simulink model "Lab2_Task_5_final"  (R2025a)
settings: Solver=FixedStepAuto  StartTime=0.0  StopTime=inf  RelTol=1e-3
model workspace (MAT data in the model file):
  SL_ROS_VariableLengthArrays_MaxSizes.CommonInfo.ArrayTruncateAction = 'EmitWarning'
  SL_ROS_VariableLengthArrays_MaxSizes.MsgTypeMap = containers.Map
  SL_ROS_VariableLengthArrays_MaxSizes.MsgTypeMap.serialization.keys = {'sensor_msgs/LaserScan'}
  SL_ROS_VariableLengthArrays_MaxSizes.MsgTypeMap.serialization.values{1}(1).PropertyName = 'intensities'
  SL_ROS_VariableLengthArrays_MaxSizes.MsgTypeMap.serialization.values{1}(1).DataType = 'single'
  SL_ROS_VariableLengthArrays_MaxSizes.MsgTypeMap.serialization.values{1}(1).MaxLength = 360
  SL_ROS_VariableLengthArrays_MaxSizes.MsgTypeMap.serialization.values{1}(2).PropertyName = 'ranges'
  SL_ROS_VariableLengthArrays_MaxSizes.MsgTypeMap.serialization.values{1}(2).DataType = 'single'
  SL_ROS_VariableLengthArrays_MaxSizes.MsgTypeMap.serialization.values{1}(2).MaxLength = 360
  SL_ROS_VariableLengthArrays_MaxSizes.MsgTypeMap.serialization.uniformity = 0
  SL_ROS_VariableLengthArrays_MaxSizes.MsgTypeMap.serialization.keyType = 'char'
  SL_ROS_VariableLengthArrays_MaxSizes.MsgTypeMap.serialization.valueType = 'any'
undefined symbols (not defined in the file or in its folder): angdiff, header, twist
libraries: ros2lib x4, simulink_extras x1, simulink x1
(part 1 of 2)
settings Model: Creator=scott  LastModifiedBy=abodynasser22
settings OptimizationCC: DefaultParameterBehavior=Inlined  EnhancedBackFolding=on  PassReuseOutputArgsAs=Individual arguments  ZeroExternalMemoryAtStartup=off  ZeroInternalMemoryAtStartup=off  MaxStackSize=64  OptimizeBlockOrder=speed  DifferentSizesBufferReuse=on  OptimizationCustomize=off  EfficientTunableParamExpr=on
settings DebuggingCC: ParameterTunabilityLossMsg=error
settings HardwareCC: ProdBitPerPointer=32.0  ProdBitPerSizeT=32.0  ProdBitPerPtrDiffT=32.0  ProdWordSize=32.0  ProdHWDeviceType=Intel->x86-32 (Windows32)  UseEmbeddedCoderFeatures=off
settings SFSimCC: MATLABDynamicMemAlloc=off
settings RTWCC: SystemTargetFile=ert.tlc  HardwareBoard=Robot Operating System 2 (ROS 2)  TLCOptions="-aInlineSetEventsForThisBaseRateFcn=TLC_FALSE -aSuppressMultiTaskScheduler=TLC_FALSE  -aRateBasedStepFcn=0"  TemplateMakefile=ert_default_tmf  Toolchain=Colcon Tools  TargetLang=C++  Description=Embedded Coder
settings CodeAppCC: ForceParamTrailComments=on  IgnoreCustomStorageClasses=off  OperatorAnnotations=on  SimulinkDataObjDesc=on  SFDataObjDesc=on  InsertBlockDesc=on
settings ERTTargetCC: ExtModeTransport=2.0  ExtModeAutomaticAllocSize=off  RootIOFormat=Structure reference  CodeInterfacePackaging=C++ class  SupportNonInlinedSFcns=on

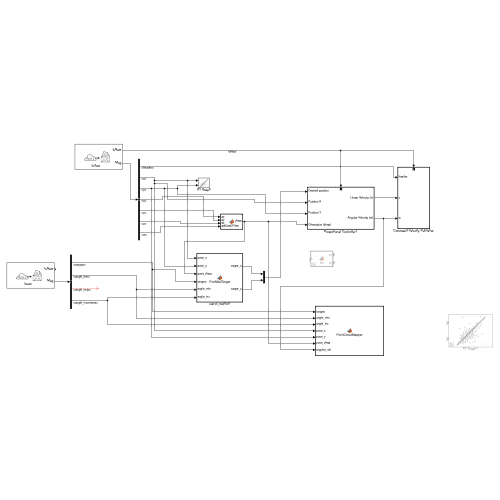
[thumbnail: Simulink's stored preview of the top-level diagram]
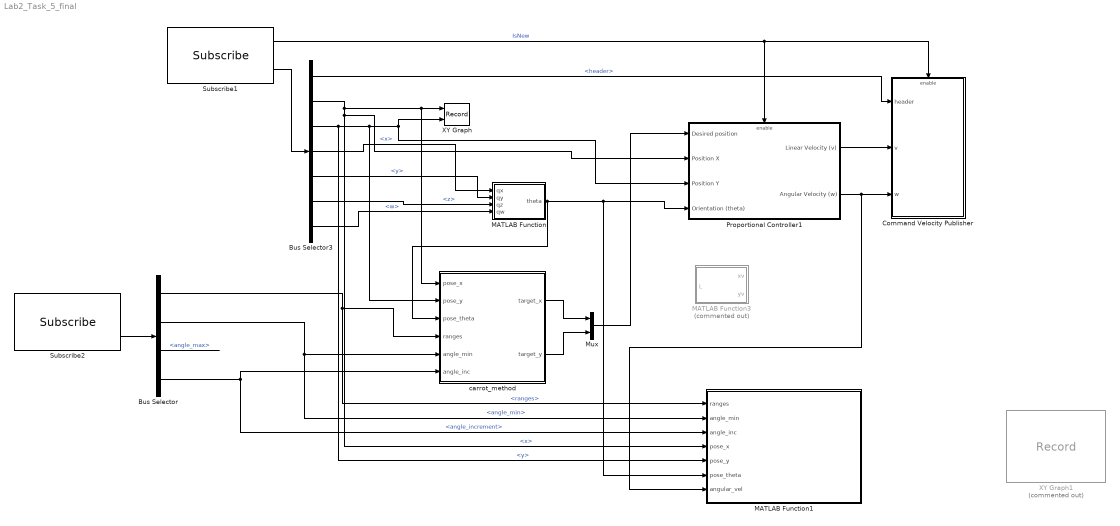
== system Lab2_Task_5_final ==
  Bus Selector : BusSelector  OutputSignals=ranges,angle_min,angle_max,angle_increment
  Bus Selector3 : BusSelector  OutputSignals=header,pose.pose.position.x,pose.pose.position.y,pose.pose.orientation.x,pose.pose.orientation.y,pose.pose.orientation.z,pose.pose.orientation.w
  Command Velocity Publisher : Subsystem
  MATLAB Function : MATLAB Function  TreatAsAtomicUnit=on
  MATLAB Function1 : MATLAB Function  TreatAsAtomicUnit=on
  MATLAB Function3 : MATLAB Function  Commented=on  TreatAsAtomicUnit=on
  Mux : Mux  Inputs=2
  Proportional Controller1 : Subsystem
  Subscribe1 : ros2lib/Subscribe  topicSource=Select from ROS network  topic=/odom  messageType=nav_msgs/Odometry  sampleTime=-1  QOSHistory=Keep last  QOSDepth=10  QOSReliability=Reliable  QOSDurability=Volatile  QOSDeadline=Inf  QOSLifespan=Inf  QOSLiveliness=Automatic  QOSLeaseDuration=Inf  QOSAvoidROSNamespaceConventions=off
  Subscribe2 : ros2lib/Subscribe  topicSource=Select from ROS network  topic=/scan  messageType=sensor_msgs/LaserScan  sampleTime=-1  QOSHistory=Keep last  QOSDepth=10  QOSReliability=Best effort  QOSDurability=Volatile  QOSDeadline=Inf  QOSLifespan=Inf  QOSLiveliness=Automatic  QOSLeaseDuration=Inf  QOSAvoidROSNamespaceConventions=off
  XY Graph : Record  NumPorts=2.0  FileSettingsInternal="{\"entries\":[{\"content\":{\"excelSettings\":{\"content\":{},\"type\":\"Streamout.ExcelSettings\"},\"parquetSettings\":{\"content\":{},\"type\":\"Streamout.ParquetSettings\"}},\"type\":\"Streamout.FileSettingStorage\",\"uuid\":\"\"}],\"packageUris\":[\"http:\\/\\/schema.mathworks.com\\/mf0\\/streamout_blocks\\/R2020a\"],\"version\":\"1.0\"}"  FrameSettings=[0, 0]  Layout=[1 1]  SignalsInternal="{\"entries\":[{\"content\":{\"signals\":[{\"content\":{\"blockPath\":[],\"dimensions\":[1],\"domain\":\"\",\"lineColor\":\"#b746ff\",\"lineWidth\":2,\"port\":1,\"signalID\":1,\"signalName\":\"<x>\"},\"type\":\"RecordBlkView.Signal\",\"uuid\":\"\"},{\"content\":{\"blockPath\":[],\"dimensions\":[1],\"domain\":\"\",\"lineColor\":\"#64d413\",\"lineWidth\":2,\"port\":2,\"signalID\":2,\"signalName\":\"<y>\"},\"type\":\"RecordBlkView.Signal\",\"uuid\":\"\"}]},\"type\":\"RecordBlkView.InputSignals\",\"uuid\":\"\"}],\"packageUris\":[\"http:\\/\\/schema.mathworks.com\\/mf0\\/streamout_blocks\\/R2020a\"],\"version\":\"1.0\"}"  VisualizationBindings="{\"xyplotplugin\":{\"info\":[{\"series\":[],\"subplotID\":1}]}}"  CompatibilityTag=XY
  XY Graph1 : Record  Commented=on  NumPorts=2.0  FileSettingsInternal="{\"entries\":[{\"content\":{\"excelSettings\":{\"content\":{},\"type\":\"Streamout.ExcelSettings\"},\"parquetSettings\":{\"content\":{},\"type\":\"Streamout.ParquetSettings\"}},\"type\":\"Streamout.FileSettingStorage\",\"uuid\":\"\"}],\"packageUris\":[\"http:\\/\\/schema.mathworks.com\\/mf0\\/streamout_blocks\\/R2020a\"],\"version\":\"1.0\"}"  FrameSettings=[0, 0]  Layout=[1 1]  SignalsInternal="{\"entries\":[{\"content\":{\"signals\":[{\"content\":{\"blockPath\":[],\"dimensions\":[360,1],\"domain\":\"\",\"hasChildren\":true,\"lineColor\":\"#d95319\",\"lineWidth\":2,\"port\":1,\"signalID\":1,\"signalName\":\"MATLAB Function1:1\"},\"type\":\"RecordBlkView.Signal\",\"uuid\":\"\"},{\"content\":{\"blockPath\":[],\"channel\":[1,1],\"dimensions\":[360,1],\"domain\":\"\",\"lineColor\":\"#edb120\",\"lineWidth\":2,\"parentID\":1,\"plots\":[ 1 ],\"port\":1,\"signalID\":2,\"signalName\":\"MATLAB Function1:1\"},\"type\":\"RecordBlkView.Signal\",\"uuid\":\"\"},{\"content\":{\"blockPath\":[],\"channel\":[2,1],\"dimensions\":[360,1],\"domain\":\"\",\"lineColor\":\"#a2142f\",\"lineWidth\":2,\"parentID\":1,\"port\":1,\"signalID\":3,\"signalName\":\"MATLAB Function1:1\"},\"type\":\"RecordBlkView.Signal\",\"uuid\":\"\"},{\"content\":{\"blockPath\":[],\"channel\":[3,1],\"dimensions\":[360,1],\"domain\":\"\",\"lineColor\":\"#139fff\",\"lineWidth\":2,\"parentID\":1,\"port\":1,\"signalID\":4,\"signalName\":\"MATLAB Function1:1\"},\"type\":\"RecordBlkView.Signal\",\"uuid\":\"\"},{\"content\":{\"blockPath\":[],\"channel\":[4,1],\"dimensions\":[360,1],\"domain\":\"\",\"lineColor\":\"#ff6929\",\"lineWidth\":2,\"parentID\":1,\"port\":1,\"signalID\":5,\"signalName\":\"MATLAB Function1:1\"},\"type\":\"RecordBlkView.Signal\",\"uuid\":\"\"},{\"content\":{\"blockPath\":[],\"channel\":[5,1],\"dimensions\":[360,1],\"domain\":\"\",\"lineColor\":\"#b746ff\",\"lineWidth\":2,\"parentID\":1,\"port\":1,\"signalID\":6,\"signalName\":\"MATLAB Function1:1\"},\"type\":\"RecordBlkView.Signal\",\"uuid\":\"\"},{\"content\":{\"blockPath\":[],\"channel\":[6,1],\"dimensions\":[360,1],\"domain\":\"\",\"lineColor\":\"#64d413\",\"lineWidth\":2,\"parentID\":1,\"port\":1,\"signalID\":7,\"signalName\":\"MATLAB Function1:1\"},\"type\":\"RecordBlkView.Signal\",\"uuid\":\"\"},{\"content\":{\"blockPath\":[],\"channel\":[7,1],\"dimensions\":[360,1],\"domain\":\"\",\"lineColor\":\"#ff13a6\",\"lineWidth\":2,\"parentID\":1,\"port\":1,\"signalID\":8,\"signalName\":\"MATLAB Function1:1\"},\"type\":\"RecordBlkView.Signal\",\"uuid\":\"\"},{\"content\":{\"blockPath\":[],\"channel\":[8,1],\"dimensions\":[360,1],\"domain\":\"\",\"lineColor\":\"#fe330a\",\"lineWidth\":2,\"parentID\":1,\"port\":1,\"signalID\":9,\"signalName\":\"MATLAB Function1:1\"},\"type\":\"RecordBlkView.Signal\",\"uuid\":\"\"},{\"content\":{\"blockPath\":[],\"channel\":[9,1],\"dimensions\":[360,1],\"domain\":\"\",\"lineColor\":\"#22b573\",\"lineWidth\":2,\"parentID\":1,\"port\":1,\"signalID\":10,\"signalName\":\"MATLAB Function1:1\"},\"type\":\"RecordBlkView.Signal\",\"uuid\":\"\"},{\"content\":{\"blockPath\":[],\"channel\":[10,1],\"dimensions\":[360,1],\"domain\":\"\",\"lineColor\":\"#0072bd\",\"lineWidth\":2,\"parentID\":1,\"port\":1,\"signalID\":11,\"signalName\":\"MATLAB Function1:1\"},\"type\":\"RecordBlkView.Signal\",\"uuid\":\"\"},{\"content\":{\"blockPath\":[],\"channel\":[11,1],\"dimensions\":[360,1],\"domain\":\"\",\"lineColor\":\"#d95319\",\"lineWidth\":2,\"parentID\":1,\"port\":1,\"signalID\":12,\"signalName\":\"MATLAB Function1:1\"},\"type\":\"RecordBlkView.Signal\",\"uuid\":\"\"},{\"content\":{\"blockPath\":[],\"channel\":[12,1],\"dimensions\":[360,1],\"domain\":\"\",\"lineColor\":\"#edb120\",\"lineWidth\":2,\"parentID\":1,\"port\":1,\"signalID\":13,\"signalName\":\"MATLAB Function1:1\"},\"type\":\"RecordBlkView.Signal\",\"uuid\":\"\"},{\"content\":{\"blockPath\":[],\"channel\":[13,1],\"dimensions\":[360,1],\"domain\":\"\",\"lineColor\":\"#7e2f8e\",\"lineWidth\":2,\"parentID\":1,\"port\":1,\"signalID\":14,\"signalName\":\"MATLAB Function1:1\"},\"type\":\"RecordBlkView.Signal\",\"uuid\":\"\"},{\"content\":{\"blockPath\":[],\"channel\":[14,1],\"dimensions\":[360,1],\"domain\":\"\",\"lineColor\":\"#77ac30\",\"lineWidth\":2,\"parentID\":1,\"port\":1,\"signalID\":15,\"signalName\":\"MATLAB Function1:1\"},\"type\":\"RecordBlkView.Signal\",\"uuid\":\"\"},{\"content\":{\"blockPath\":[],\"channel\":[15,1],\"dimensions\":[360,1],\"domain\":\"\",\"lineColor\":\"#4dbeee\",\"lineWidth\":2,\"parentID\":1,\"port\":1,\"signalID\":16,\"signalName\":\"MATLAB Function1:1\"},\"type\":\"RecordBlkView.Signal\",\"uuid\":\"\"},{\"content\":{\"blockPath\":[],\"channel\":[16,1],\"dimensions\":[360,1],\"domain\":\"\",\"lineColor\":\"#a2142f\",\"lineWidth\":2,\"parentID\":1,\"port\":1,\"signalID\":17,\"signalName\":\"MATLAB Function1:1\"},\"type\":\"RecordBlkView.Signal\",\"uuid\":\"\"},{\"content\":{\"blockPath\":[],\"channel\":[17,1],\"dimensions\":[360,1],\"domain\":\"\",\"lineColor\":\"#139fff\",\"lineWidth\":2,\"parentID\":1,\"port\":1,\"signalID\":18,\"signalName\":\"MATLAB Function1:1\"},\"type\":\"RecordBlkView.Signal\",\"uuid\":\"\"},{\"content\":{\"blockPath\":[],\"channel\":[18,1],\"dimensions\":[360,1],\"domain\":\"\",\"lineColor\":\"#ff6929\",\"lineWidth\":2,\"parentID\":1,\"port\":1,\"signalID\":19,\"signalName\":\"MATLAB Function1:1\"},\"type\":\"RecordBlkView.Signal\",\"uuid\":\"\"},{\"content\":{\"blockPath\":[],\"channel\":[19,1],\"dimensions\":[360,1],\"domain\":\"\",\"lineColor\":\"#b746ff\",\"lineWidth\":2,\"parentID\":1,\"port\":1,\"signalID\":20,\"signalName\":\"MATLAB Function1:1\"},\"type\":\"RecordBlkView.Signal\",\"uuid\":\"\"},{\"content\":{\"blockPath\":[],\"channel\":[20,1],\"dimensions\":[360,1],\"domain\":\"\",\"lineColor\":\"#64d413\",\"lineWidth\":2,\"parentID\":1,\"port\":1,\"signalID\":21,\"signalName\":\"MATLAB Function1:1\"},\"type\":\"RecordBlkView.Signal\",\"uuid\":\"\"},{\"content\":{\"blockPath\":[],\"channel\":[21,1],\"dimensions\":[360,1],\"domain\":\"\",\"lineColor\":\"#ff13a6\",\"lineWidth\":2,\"parentID\":1,\"port\":1,\"signalID\":22,\"signalName\":\"MATLAB Function1:1\"},\"type\":\"RecordBlkView.Signal\",\"uuid\":\"\"},{\"content\":{\"blockPath\":[],\"channel\":[22,1],\"dimensions\":[360,1],\"domain\":\"\",\"lineColor\":\"#fe330a\",\"lineWidth\":2,\"parentID\":1,\"port\":1,\"signalID\":23,\"signalName\":\"MATLAB Function1:1\"},\"type\":\"RecordBlkView.Signal\",\"uuid\":\"\"},{\"content\":{\"blockPath\":[],\"channel\":[23,1],\"dimensions\":[360,1],\"domain\":\"\",\"lineColor\":\"#22b573\",\"lineWidth\":2,\"parentID\":1,\"port\":1,\"signalID\":24,\"signalName\":\"MATLAB Function1:1\"},\"type\":\"RecordBlkView.Signal\",\"uuid\":\"\"},{\"content\":{\"blockPath\":[],\"channel\":[24,1],\"dimensions\":[360,1],\"domain\":\"\",\"lineColor\":\"#0072bd\",\"lineWidth\":2,\"parentID\":1,\"port\":1,\"signalID\":25,\"signalName\":\"MATLAB Function1:1\"},\"type\":\"RecordBlkView.Signal\",\"uuid\":\"\"},{\"content\":{\"blockPath\":[],\"channel\":[25,1],\"dimensions\":[360,1],\"domain\":\"\",\"lineColor\":\"#d95319\",\"lineWidth\":2,\"parentID\":1,\"port\":1,\"signalID\":26,\"signalName\":\"MATLAB Function1:1\"},\"type\":\"RecordBlkView.Signal\",\"uuid\":\"\"},{\"content\":{\"blockPath\":[],\"channel\":[26,1],\"dimensions\":[360,1],\"domain\":\"\",\"lineColor\":\"#edb120\",\"lineWidth\":2,\"parentID\":1,\"port\":1,\"signalID\":27,\"signalName\":\"MATLAB Function1:1\"},\"type\":\"RecordBlkView.Signal\",\"uuid\":\"\"},{\"content\":{\"blockPath\":[],\"channel\":[27,1],\"dimensions\":[360,1],\"domain\":\"\",\"lineColor\":\"#7e2f8e\",\"lineWidth\":2,\"parentID\":1,\"port\":1,\"signalID\":28,\"signalName\":\"MATLAB Function1:1\"},\"type\":\"RecordBlkView.Signal\",\"uuid\":\"\"},{\"content\":{\"blockPath\":[],\"channel\":[28,1],\"dimensions\":[360,1],\"domain\":\"\",\"lineColor\":\"#77ac30\",\"lineWidth\":2,\"parentID\":1,\"port\":1,\"signalID\":29,\"signalName\":\"MATLAB Function1:1\"},\"type\":\"RecordBlkView.Signal\",\"uuid\":\"\"},{\"content\":{\"blockPath\":[],\"channel\":[29,1],\"dimensions\":[360,1],\"domain\":\"\",\"lineColor\":\"#4dbeee\",\"lineWidth\":2,\"parentID\":1,\"port\":1,\"signalID\":30,\"signalName\":\"MATLAB Function1:1\"},\"type\":\"RecordBlkView.Signal\",\"uuid\":\"\"},{\"content\":{\"blockPath\":[],\"channel\":[30,1],\"dimensions\":[360,1],\"domain\":\"\",\"lineColor\":\"#a2142f\",\"lineWidth\":2,\"parentID\":1,\"port\":1,\"signalID\":31,\"signalName\":\"MATLAB Function1:1\"},\"type\":\"RecordBlkView.Signal\",\"uuid\":\"\"},{\"content\":{\"blockPath\":[],\"channel\":[31,1],\"dimensions\":[360,1],\"domain\":\"\",\"lineColor\":\"#139fff\",\"lineWidth\":2,\"parentID\":1,\"port\":1,\"signalID\":32,\"signalName\":\"MATLAB Function1:1\"},\"type\":\"RecordBlkView.Signal\",\"uuid\":\"\"},{\"content\":{\"blockPath\":[],\"channel\":[32,1],\"dimensions\":[360,1],\"domain\":\"\",\"lineColor\":\"#ff6929\",\"lineWidth\":2,\"parentID\":1,\"port\":1,\"signalID\":33,\"signalName\":\"MATLAB Function1:1\"},\"type\":\"RecordBlkView.Signal\",\"uuid\":\"\"},{\"content\":{\"blockPath\":[],\"channel\":[33,1],\"dimensions\":[360,1],\"domain\":\"\",\"lineColor\":\"#b746ff\",\"lineWidth\":2,\"parentID\":1,\"port\":1,\"signalID\":34,\"signalName\":\"MATLAB Function1:1\"},\"type\":\"RecordBlkView.Signal\",\"uuid\":\"\"},{\"content\":{\"blockPath\":[],\"channel\":[34,1],\"dimensions\":[360,1],\"domain\":\"\",\"lineColor\":\"#64d413\",\"lineWidth\":2,\"parentID\":1,\"port\":1,\"signalID\":35,\"signalName\":\"MATLAB Function1:1\"},\"type\":\"RecordBlkView.Signal\",\"uuid\":\"\"},{\"content\":{\"blockPath\":[],\"channel\":[35,1],\"dimensions\":[360,1],\"domain\":\"\",\"lineColor\":\"#ff13a6\",\"lineWidth\":2,\"parentID\":1,\"port\":1,\"signalID\":36,\"signalName\":\"MATLAB Function1:1\"},\"type\":\"RecordBlkView.Signal\",\"uuid\":\"\"},{\"content\":{\"blockPath\":[],\"channel\":[36,1],\"dimensions\":[360,1],\"domain\":\"\",\"lineColor\":\"#fe330a\",\"lineWidth\":2,\"parentID\":1,\"port\":1,\"signalID\":37,\"signalName\":\"MATLAB Function1:1\"},\"type\":\"RecordBlkView.Signal\",\"uuid\":\"\"},{\"content\":{\"blockPath\":[],\"channel\":[37,1],\"dimensions\":[360,1],\"domain\":\"\",\"lineColor\":\"#22b573\",\"lineWidth\":2,\"parentID\":1,\"port\":1,\"signalID\":38,\"signalName\":\"MATLAB Function1:1\"},\"type\":\"RecordBlkView.Signal\",\"uuid\":\"\"},{\"content\":{\"blockPath\":[],\"channel\":[38,1],\"dimensions\":[360,1],\"domain\":\"\",\"lineColor\":\"#0072bd\",\"lineWidth\":2,\"parentID\":1,\"port\":1,\"signalID\":39,\"signalName\":\"MATLAB Function1:1\"},\"type\":\"RecordBlkView.Signal\",\"uuid\":\"\"},{\"content\":{\"blockPath\":[],\"channel\":[39,1],\"dimensions\":[360,1],\"domain\":\"\",\"lineColor\":\"#d95319\",\"lineWidth\":2,\"parentID\":1,\"port\":1,\"signalID\":40,\"signalName\":\"MATLAB Function1:1\"},\"type\":\"RecordBlkView.Signal\",\"uuid\":\"\"},{\"content\":{\"blockPath\":[],\"channel\":[40,1],\"dimensions\":[360,1],\"domain\":\"\",\"lineColor\":\"#edb120\",\"lineWidth\":2,\"parentID\":1,\"port\":1,\"signalID\":41,\"signalName\":\"MATLAB Function1:1\"},\"type\":\"RecordBlkView.Signal\",\"uuid\":\"\"},{\"content\":{\"blockPath\":[],\"channel\":[41,1],\"dimensions\":[360,1],\"domain\":\"\",\"lineColor\":\"#7e2f8e\",\"lineWidth\":2,\"parentID\":1,\"port\":1,\"signalID\":42,\"signalName\":\"MATLAB Function1:1\"},\"type\":\"RecordBlkView.Signal\",\"uuid\":\"\"},{\"content\":{\"blockPath\":[],\"channel\":[42,1],\"dimensions\":[360,1],\"domain\":\"\",\"lineColor\":\"#77ac30\",\"lineWidth\":2,\"parentID\":1,\"port\":1,\"signalID\":43,\"signalName\":\"MATLAB Function1:1\"},\"type\":\"RecordBlkView.Signal\",\"uuid\":\"\"},{\"content\":{\"blockPath\":[],\"channel\":[43,1],\"dimensions\":[360,1],\"domain\":\"\",\"lineColor\":\"#4dbeee\",\"lineWidth\":2,\"parentID\":1,\"port\":1,\"signalID\":44,\"signalName\":\"MATLAB Function1:1\"},\"type\":\"RecordBlkView.Signal\",\"uuid\":\"\"},{\"content\":{\"blockPath\":[],\"channel\":[44,1],\"dimensions\":[360,1],\"domain\":\"\",\"lineColor\":\"#a2142f\",\"lineWidth\":2,\"parentID\":1,\"port\":1,\"signalID\":45,\"signalName\":\"MATLAB Function1:1\"},\"type\":\"RecordBlkView.Signal\",\"uuid\":\"\"},{\"content\":{\"blockPath\":[],\"channel\":[45,1],\"dimensions\":[360,1],\"domain\":\"\",\"lineColor\":\"#139fff\",\"lineWidth\":2,\"parentID\":1,\"port\":1,\"signalID\":46,\"signalName\":\"MATLAB Function1:1\"},\"type\":\"RecordBlkView.Signal\",\"uuid\":\"\"},{\"content\":{\"blockPath\":[],\"channel\":[46,1],\"dimensions\":[360,1],\"domain\":\"\",\"lineColor\":\"#ff6929\",\"lineWidth\":2,\"parentID\":1,\"port\":1,\"signalID\":47,\"signalName\":\"MATLAB Function1:1\"},\"type\":\"RecordBlkView.Signal\",\"uuid\":\"\"},{\"content\":{\"blockPath\":[],\"channel\":[47,1],\"dimensions\":[360,1],\"domain\":\"\",\"lineColor\":\"#b746ff\",\"lineWidth\":2,\"parentID\":1,\"port\":1,\"signalID\":48,\"signalName\":\"MATLAB Function1:1\"},\"type\":\"RecordBlkView.Signal\",\"uuid\":\"\"},{\"content\":{\"blockPath\":[],\"channel\":[48,1],\"dimensions\":[360,1],\"domain\":\"\",\"lineColor\":\"#64d413\",\"lineWidth\":2,\"parentID\":1,\"port\":1,\"signalID\":49,\"signalName\":\"MATLAB Function1:1\"},\"type\":\"RecordBlkView.Signal\",\"uuid\":\"\"},{\"content\":{\"blockPath\":[],\"channel\":[49,1],\"dimensions\":[360,1],\"domain\":\"\",\"lineColor\":\"#ff13a6\",\"lineWidth\":2,\"parentID\":1,\"port\":1,\"signalID\":50,\"signalName\":\"MATLAB Function1:1\"},\"type\":\"RecordBlkView.Signal\",\"uuid\":\"\"},{\"content\":{\"blockPath\":[],\"channel\":[50,1],\"dimensions\":[360,1],\"domain\":\"\",\"lineColor\":\"#fe330a\",\"lineWidth\":2,\"parentID\":1,\"port\":1,\"signalID\":51,\"signalName\":\"MATLAB Function1:1\"},\"type\":\"RecordBlkView.Signal\",\"uuid\":\"\"},{\"content\":{\"blockPath\":[],\"channel\":[51,1],\"dimensions\":[360,1],\"domain\":\"\",\"lineColor\":\"#22b573\",\"lineWidth\":2,\"parentID\":1,\"port\":1,\"signalID\":52,\"signalName\":\"MATLAB Function1:1\"},\"type\":\"RecordBlkView.Signal\",\"uuid\":\"\"},{\"content\":{\"blockPath\":[],\"channel\":[52,1],\"dimensions\":[360,1],\"domain\":\"\",\"lineColor\":\"#0072bd\",\"lineWidth\":2,\"parentID\":1,\"port\":1,\"signalID\":53,\"signalName\":\"MATLAB Function1:1\"},\"type\":\"RecordBlkView.Signal\",\"uuid\":\"\"},{\"content\":{\"blockPath\":[],\"channel\":[53,1],\"dimensions\":[360,1],\"domain\":\"\",\"lineColor\":\"#d95319\",\"lineWidth\":2,\"parentID\":1,\"port\":1,\"signalID\":54,\"signalName\":\"MATLAB Function1:1\"},\"type\":\"RecordBlkView.Signal\",\"uuid\":\"\"},{\"content\":{\"blockPath\":[],\"channel\":[54,1],\"dimensions\":[360,1],\"domain\":\"\",\"lineColor\":\"#edb120\",\"lineWidth\":2,\"parentID\":1,\"port\":1,\"signalID\":55,\"signalName\":\"MATLAB Function1:1\"},\"type\":\"RecordBlkView.Signal\",\"uuid\":\"\"},{\"content\":{\"blockPath\":[],\"channel\":[55,1],\"dimensions\":[360,1],\"domain\":\"\",\"lineColor\":\"#7e2f8e\",\"lineWidth\":2,\"parentID\":1,\"port\":1,\"signalID\":56,\"signalName\":\"MATLAB Function1:1\"},\"type\":\"RecordBlkView.Signal\",\"uuid\":\"\"},{\"content\":{\"blockPath\":[],\"channel\":[56,1],\"dimensions\":[360,1],\"domain\":\"\",\"lineColor\":\"#77ac30\",\"lineWidth\":2,\"parentID\":1,\"port\":1,\"signalID\":57,\"signalName\":\"MATLAB Function1:1\"},\"type\":\"RecordBlkView.Signal\",\"uuid\":\"\"},{\"content\":{\"blockPath\":[],\"channel\":[57,1],\"dimensions\":[360,1],\"domain\":\"\",\"lineColor\":\"#4dbeee\",\"lineWidth\":2,\"parentID\":1,\"port\":1,\"signalID\":58,\"signalName\":\"MATLAB Function1:1\"},\"type\":\"RecordBlkView.Signal\",\"uuid\":\"\"},{\"content\":{\"blockPath\":[],\"channel\":[58,1],\"dimensions\":[360,1],\"domain\":\"\",\"lineColor\":\"#a2142f\",\"lineWidth\":2,\"parentID\":1,\"port\":1,\"signalID\":59,\"signalName\":\"MATLAB Function1:1\"},\"type\":\"RecordBlkView.Signal\",\"uuid\":\"\"},{\"content\":{\"blockPath\":[],\"channel\":[59,1],\"dimensions\":[360,1],\"domain\":\"\",\"lineColor\":\"#139fff\",\"lineWidth\":2,\"parentID\":1,\"port\":1,\"signalID\":60,\"signalName\":\"MATLAB Function1:1\"},\"type\":\"RecordBlkView.Signal\",\"uuid\":\"\"},{\"content\":{\"blockPath\":[],\"channel\":[60,1],\"dimensions\":[360,1],\"domain\":\"\",\"lineColor\":\"#ff6929\",\"lineWidth\":2,\"parentID\":1,\"port\":1,\"signalID\":61,\"signalName\":\"MATLAB Function1:1\"},\"type\":\"RecordBlkView.Signal\",\"uuid\":\"\"},{\"content\":{\"blockPath\":[],\"channel\":[61,1],\"dimensions\":[360,1],\"domain\":\"\",\"lineColor\":\"#b746ff\",\"lineWidth\":2,\"parentID\":1,\"port\":1,\"signalID\":62,\"signalName\":\"MATLAB Function1:1\"},\"type\":\"RecordBlkView.Signal\",\"uuid\":\"\"},{\"content\":{\"blockPath\":[],\"channel\":[62,1],\"dimensions\":[360,1],\"domain\":\"\",\"lineColor\":\"#64d413\",\"lineWidth\":2,\"parentID\":1,\"port\":1,\"signalID\":63,\"signalName\":\"MATLAB Function1:1\"},\"type\":\"RecordBlkView.Signal\",\"uuid\":\"\"},{\"content\":{\"blockPath\":[],\"channel\":[63,1],\"dimensions\":[360,1],\"domain\":\"\",\"lineColor\":\"#ff13a6\",\"lineWidth\":2,\"parentID\":1,\"port\":1,\"signalID\":64,\"signalName\":\"MATLAB Function1:1\"},\"type\":\"RecordBlkView.Signal\",\"uuid\":\"\"},{\"content\":{\"blockPath\":[],\"channel\":[64,1],\"dimensions\":[360,1],\"domain\":\"\",\"lineColor\":\"#fe330a\",\"lineWidth\":2,\"parentID\":1,\"port\":1,\"signalID\":65,\"signalName\":\"MATLAB Function1:1\"},\"type\":\"RecordBlkView.Signal\",\"uuid\":\"\"},{\"content\":{\"blockPath\":[],\"channel\":[65,1],\"dimensions\":[360,1],\"domain\":\"\",\"lineColor\":\"#22b573\",\"lineWidth\":2,\"parentID\":1,\"port\":1,\"signalID\":66,\"signalName\":\"MATLAB Function1:1\"},\"type\":\"RecordBlkView.Signal\",\"uuid\":\"\"},{\"content\":{\"blockPath\":[],\"channel\":[66,1],\"dimensions\":[360,1],\"domain\":\"\",\"lineColor\":\"#0072bd\",\"lineWidth\":2,\"parentID\":1,\"port\":1,\"signalID\":67,\"signalName\":\"MATLAB Function1:1\"},\"type\":\"RecordBlkView.Signal\",\"uuid\":\"\"},{\"content\":{\"blockPath\":[],\"channel\":[67,1],\"dimensions\":[360,1],\"domain\":\"\",\"lineColor\":\"#d95319\",\"lineWidth\":2,\"parentID\":1,\"port\":1,\"signalID\":68,\"signalName\":\"MATLAB Function1:1\"},\"type\":\"RecordBlkView.Signal\",\"uuid\":\"\"},{\"content\":{\"blockPath\":[],\"channel\":[68,1],\"dimensions\":[360,1],\"domain\":\"\",\"lineColor\":\"#edb120\",\"lineWidth\":2,\"parentID\":1,\"port\":1,\"signalID\":69,\"signalName\":\"MATLAB Function1:1\"},\"type\":\"RecordBlkView.Signal\",\"uuid\":\"\"},{\"content\":{\"blockPath\":[],\"channel\":[69,1],\"dimensions\":[360,1],\"domain\":\"\",\"lineColor\":\"#7e2f8e\",\"lineWidth\":2,\"parentID\":1,\"port\":1,\"signalID\":70,\"signalName\":\"MATLAB Function1:1\"},\"type\":\"RecordBlkView.Signal\",\"uuid\":\"\"},{\"content\":{\"blockPath\":[],\"channel\":[70,1],\"dimensions\":[360,1],\"domain\":\"\",\"lineColor\":\"#77ac30\",\"lineWidth\":2,\"parentID\":1,\"port\":1,\"signalID\":71,\"signalName\":\"MATLAB Function1:1\"},\"type\":\"RecordBlkView.Signal\",\"uuid\":\"\"},{\"content\":{\"blockPath\":[],\"channel\":[71,1],\"dimensions\":[360,1],\"domain\":\"\",\"lineColor\":\"#4dbeee\",\"lineWidth\":2,\"parentID\":1,\"port\":1,\"signalID\":72,\"signalName\":\"MATLAB Function1:1\"},\"type\":\"RecordBlkView.Signal\",\"uuid\":\"\"},{\"content\":{\"blockPath\":[],\"channel\":[72,1],\"dimensions\":[360,1],\"domain\":\"\",\"lineColor\":\"#a2142f\",\"lineWidth\":2,\"parentID\":1,\"port\":1,\"signalID\":73,\"signalName\":\"MATLAB Function1:1\"},\"type\":\"RecordBlkView.Signal\",\"uuid\":\"\"},{\"content\":{\"blockPath\":[],\"channel\":[73,1],\"dimensions\":[360,1],\"domain\":\"\",\"lineColor\":\"#139fff\",\"lineWidth\":2,\"parentID\":1,\"port\":1,\"signalID\":74,\"signalName\":\"MATLAB Function1:1\"},\"type\":\"RecordBlkView.Signal\",\"uuid\":\"\"},{\"content\":{\"blockPath\":[],\"channel\":[74,1],\"dimensions\":[360,1],\"domain\":\"\",\"lineColor\":\"#ff6929\",\"lineWidth\":2,\"parentID\":1,\"port\":1,\"signalID\":75,\"signalName\":\"MATLAB Function1:1\"},\"type\":\"RecordBlkView.Signal\",\"uuid\":\"\"},{\"content\":{\"blockPath\":[],\"channel\":[75,1],\"dimensions\":[360,1],\"domain\":\"\",\"lineColor\":\"#b746ff\",\"lineWidth\":2,\"parentID\":1,\"port\":1,\"signalID\":76,\"signalName\":\"MATLAB Function1:1\"},\"type\":\"RecordBlkView.Signal\",\"uuid\":\"\"},{\"content\":{\"blockPath\":[],\"channel\":[76,1],\"dimensions\":[360,1],\"domain\":\"\",\"lineColor\":\"#64d413\",\"lineWidth\":2,\"parentID\":1,\"port\":1,\"signalID\":77,\"signalName\":\"MATLAB Function1:1\"},\"type\":\"RecordBlkView.Signal\",\"uuid\":\"\"},{\"content\":{\"blockPath\":[],\"channel\":[77,1],\"dimensions\":[360,1],\"domain\":\"\",\"lineColor\":\"#ff13a6\",\"lineWidth\":2,\"parentID\":1,\"port\":1,\"signalID\":78,\"signalName\":\"MATLAB Function1:1\"},\"type\":\"RecordBlkView.Signal\",\"uuid\":\"\"},{\"content\":{\"blockPath\":[],\"channel\":[78,1],\"dimensions\":[360,1],\"domain\":\"\",\"lineColor\":\"#fe330a\",\"lineWidth\":2,\"parentID\":1,\"port\":1,\"signalID\":79,\"signalName\":\"MATLAB Function1:1\"},\"type\":\"RecordBlkView.Signal\",\"uuid\":\"\"},{\"content\":{\"blockPath\":[],\"channel\":[79,1],\"dimensions\":[360,1],\"domain\":\"\",\"lineColor\":\"#22b573\",\"lineWidth\":2,\"parentID\":1,\"port\":1,\"signalID\":80,\"signalName\":\"MATLAB Function1:1\"},\"type\":\"RecordBlkView.Signal\",\"uuid\":\"\"},{\"content\":{\"blockPath\":[],\"channel\":[80,1],\"dimensions\":[360,1],\"domain\":\"\",\"lineColor\":\"#0072bd\",\"lineWidth\":2,\"parentID\":1,\"port\":1,\"signalID\":81,\"signalName\":\"MATLAB Function1:1\"},\"type\":\"RecordBlkView.Signal\",\"uuid\":\"\"},{\"content\":{\"blockPath\":[],\"channel\":[81,1],\"dimensions\":[360,1],\"domain\":\"\",\"lineColor\":\"#d95319\",\"lineWidth\":2,\"parentID\":1,\"port\":1,\"signalID\":82,\"signalName\":\"MATLAB Function1:1\"},\"type\":\"RecordBlkView.Signal\",\"uuid\":\"\"},{\"content\":{\"blockPath\":[],\"channel\":[82,1],\"dimensions\":[360,1],\"domain\":\"\",\"lineColor\":\"#edb120\",\"lineWidth\":2,\"parentID\":1,\"port\":1,\"signalID\":83,\"signalName\":\"MATLAB Function1:1\"},\"type\":\"RecordBlkView.Signal\",\"uuid\":\"\"},{\"content\":{\"blockPath\":[],\"channel\":[83,1],\"dimensions\":[360,1],\"domain\":\"\",\"lineColor\":\"#7e2f8e\",\"lineWidth\":2,\"parentID\":1,\"port\":1,\"signalID\":84,\"signalName\":\"MATLAB Function1:1\"},\"type\":\"RecordBlkView.Signal\",\"uuid\":\"\"},{\"content\":{\"blockPath\":[],\"channel\":[84,1],\"dimensions\":[360,1],\"domain\":\"\",\"lineColor\":\"#77ac30\",\"lineWidth\":2,\"parentID\":1,\"port\":1,\"signalID\":85,\"signalName\":\"MATLAB Function1:1\"},\"type\":\"RecordBlkView.Signal\",\"uuid\":\"\"},{\"content\":{\"blockPath\":[],\"channel\":[85,1],\"dimensions\":[360,1],\"domain\":\"\",\"lineColor\":\"#4dbeee\",\"lineWidth\":2,\"parentID\":1,\"port\":1,\"signalID\":86,\"signalName\":\"MATLAB Function1:1\"},\"type\":\"RecordBlkView.Signal\",\"uuid\":\"\"},{\"content\":{\"blockPath\":[],\"channel\":[86,1],\"dimensions\":[360,1],\"domain\":\"\",\"lineColor\":\"#a2142f\",\"lineWidth\":2,\"parentID\":1,\"port\":1,\"signalID\":87,\"signalName\":\"MATLAB Function1:1\"},\"type\":\"RecordBlkView.Signal\",\"uuid\":\"\"},{\"content\":{\"blockPath\":[],\"channel\":[87,1],\"dimensions\":[360,1],\"domain\":\"\",\"lineColor\":\"#139fff\",\"lineWidth\":2,\"parentID\":1,\"port\":1,\"signalID\":88,\"signalName\":\"MATLAB Function1:1\"},\"type\":\"RecordBlkView.Signal\",\"uuid\":\"\"},{\"content\":{\"blockPath\":[],\"channel\":[88,1],\"dimensions\":[360,1],\"domain\":\"\",\"lineColor\":\"#ff6929\",\"lineWidth\":2,\"parentID\":1,\"port\":1,\"signalID\":89,\"signalName\":\"MATLAB Function1:1\"},\"type\":\"RecordBlkView.Signal\",\"uuid\":\"\"},{\"content\":{\"blockPath\":[],\"channel\":[89,1],\"dimensions\":[360,1],\"domain\":\"\",\"lineColor\":\"#b746ff\",\"lineWidth\":2,\"parentID\":1,\"port\":1,\"signalID\":90,\"signalName\":\"MATLAB Function1:1\"},\"type\":\"RecordBlkView.Signal\",\"uuid\":\"\"},{\"content\":{\"blockPath\":[],\"channel\":[90,1],\"dimensions\":[360,1],\"domain\":\"\",\"lineColor\":\"#64d413\",\"lineWidth\":2,\"parentID\":1,\"port\":1,\"signalID\":91,\"signalName\":\"MATLAB Function1:1\"},\"type\":\"RecordBlkView.Signal\",\"uuid\":\"\"},{\"content\":{\"blockPath\":[],\"channel\":[91,1],\"dimensions\":[360,1],\"domain\":\"\",\"lineColor\":\"#ff13a6\",\"lineWidth\":2,\"parentID\":1,\"port\":1,\"signalID\":92,\"signalName\":\"MATLAB Function1:1\"},\"type\":\"RecordBlkView.Signal\",\"uuid\":\"\"},{\"content\":{\"blockPath\":[],\"channel\":[92,1],\"dimensions\":[360,1],\"domain\":\"\",\"lineColor\":\"#fe330a\",\"lineWidth\":2,\"parentID\":1,\"port\":1,\"signalID\":93,\"signalName\":\"MATLAB Function1:1\"},\"type\":\"RecordBlkView.Signal\",\"uuid\":\"\"},{\"content\":{\"blockPath\":[],\"channel\":[93,1],\"dimensions\":[360,1],\"domain\":\"\",\"lineColor\":\"#22b573\",\"lineWidth\":2,\"parentID\":1,\"port\":1,\"signalID\":94,\"signalName\":\"MATLAB Function1:1\"},\"type\":\"RecordBlkView.Signal\",\"uuid\":\"\"},{\"content\":{\"blockPath\":[],\"channel\":[94,1],\"dimensions\":[360,1],\"domain\":\"\",\"lineColor\":\"#0072bd\",\"lineWidth\":2,\"parentID\":1,\"port\":1,\"signalID\":95,\"signalName\":\"MATLAB Function1:1\"},\"type\":\"RecordBlkView.Signal\",\"uuid\":\"\"},{\"content\":{\"blockPath\":[],\"channel\":[95,1],\"dimensions\":[360,1],\"domain\":\"\",\"lineColor\":\"#d95319\",\"lineWidth\":2,\"parentID\":1,\"port\":1,\"signalID\":96,\"signalName\":\"MATLAB Function1:1\"},\"type\":\"RecordBlkView.Signal\",\"uuid\":\"\"},{\"content\":{\"blockPath\":[],\"channel\":[96,1],\"dimensions\":[360,1],\"domain\":\"\",\"lineColor\":\"#edb120\",\"lineWidth\":2,\"parentID\":1,\"port\":1,\"signalID\":97,\"signalName\":\"MATLAB Function1:1\"},\"type\":\"RecordBlkView.Signal\",\"uuid\":\"\"},{\"content\":{\"blockPath\":[],\"channel\":[97,1],\"dimensions\":[360,1],\"domain\":\"\",\"lineColor\":\"#7e2f8e\",\"lineWidth\":2,\"parentID\":1,\"port\":1,\"signalID\":98,\"signalName\":\"MATLAB Function1:1\"},\"type\":\"RecordBlkView.Signal\",\"uuid\":\"\"},{\"content\":{\"blockPath\":[],\"channel\":[98,1],\"dimensions\":[360,1],\"domain\":\"\",\"lineColor\":\"#77ac30\",\"lineWidth\":2,\"parentID\":1,\"port\":1,\"signalID\":99,\"signalName\":\"MATLAB Function1:1\"},\"type\":\"RecordBlkView.Signal\",\"uuid\":\"\"},{\"content\":{\"blockPath\":[],\"channel\":[99,1],\"dimensions\":[360,1],\"domain\":\"\",\"lineColor\":\"#4dbeee\",\"lineWidth\":2,\"parentID\":1,\"port\":1,\"signalID\":100,\"signalName\":\"MATLAB Function1:1\"},\"type\":\"RecordBlkView.Signal\",\"uuid\":\"\"},{\"content\":{\"blockPath\":[],\"channel\":[100,1],\"dimensions\":[360,1],\"domain\":\"\",\"lineColor\":\"#a2142f\",\"lineWidth\":2,\"parentID\":1,\"port\":1,\"signalID\":101,\"signalName\":\"MATLAB Function1:1\"},\"type\":\"RecordBlkView.Signal\",\"uuid\":\"\"},{\"content\":{\"blockPath\":[],\"channel\":[101,1],\"dimensions\":[360,1],\"domain\":\"\",\"lineColor\":\"#139fff\",\"lineWidth\":2,\"parentID\":1,\"port\":1,\"signalID\":102,\"signalName\":\"MATLAB Function1:1\"},\"type\":\"RecordBlkView.Signal\",\"uuid\":\"\"},{\"content\":{\"blockPath\":[],\"channel\":[102,1],\"dimensions\":[360,1],\"domain\":\"\",\"lineColor\":\"#ff6929\",\"lineWidth\":2,\"parentID\":1,\"port\":1,\"signalID\":103,\"signalName\":\"MATLAB Function1:1\"},\"type\":\"RecordBlkView.Signal\",\"uuid\":\"\"},{\"content\":{\"blockPath\":[],\"channel\":[103,1],\"dimensions\":[360,1],\"domain\":\"\",\"lineColor\":\"#b746ff\",\"lineWidth\":2,\"parentID\":1,\"port\":1,\"signalID\":104,\"signalName\":\"MATLAB Function1:1\"},\"type\":\"RecordBlkView.Signal\",\"uuid\":\"\"},{\"content\":{\"blockPath\":[],\"channel\":[104,1],\"dimensions\":[360,1],\"domain\":\"\",\"lineColor\":\"#64d413\",\"lineWidth\":2,\"parentID\":1,\"port\":1,\"signalID\":105,\"signalName\":\"MATLAB Function1:1\"},\"type\":\"RecordBlkView.Signal\",\"uuid\":\"\"},{\"content\":{\"blockPath\":[],\"channel\":[105,1],\"dimensions\":[360,1],\"domain\":\"\",\"lineColor\":\"#ff13a6\",\"lineWidth\":2,\"parentID\":1,\"port\":1,\"signalID\":106,\"signalName\":\"MATLAB Function1:1\"},\"type\":\"RecordBlkView.Signal\",\"uuid\":\"\"},{\"content\":{\"blockPath\":[],\"channel\":[106,1],\"dimensions\":[360,1],\"domain\":\"\",\"lineColor\":\"#fe330a\",\"lineWidth\":2,\"parentID\":1,\"port\":1,\"signalID\":107,\"signalName\":\"MATLAB Function1:1\"},\"type\":\"RecordBlkView.Signal\",\"uuid\":\"\"},{\"content\":{\"blockPath\":[],\"channel\":[107,1],\"dimensions\":[360,1],\"domain\":\"\",\"lineColor\":\"#22b573\",\"lineWidth\":2,\"parentID\":1,\"port\":1,\"signalID\":108,\"signalName\":\"MATLAB Function1:1\"},\"type\":\"RecordBlkView.Signal\",\"uuid\":\"\"},{\"content\":{\"blockPath\":[],\"channel\":[108,1],\"dimensions\":[360,1],\"domain\":\"\",\"lineColor\":\"#0072bd\",\"lineWidth\":2,\"parentID\":1,\"port\":1,\"signalID\":109,\"signalName\":\"MATLAB Function1:1\"},\"type\":\"RecordBlkView.Signal\",\"uuid\":\"\"},{\"content\":{\"blockPath\":[],\"channel\":[109,1],\"dimensions\":[360,1],\"domain\":\"\",\"lineColor\":\"#d95319\",\"lineWidth\":2,\"parentID\":1,\"port\":1,\"signalID\":110,\"signalName\":\"MATLAB Function1:1\"},\"type\":\"RecordBlkView.Signal\",\"uuid\":\"\"},{\"content\":{\"blockPath\":[],\"channel\":[110,1],\"dimensions\":[360,1],\"domain\":\"\",\"lineColor\":\"#edb120\",\"lineWidth\":2,\"parentID\":1,\"port\":1,\"signalID\":111,\"signalName\":\"MATLAB Function1:1\"},\"type\":\"RecordBlkView.Signal\",\"uuid\":\"\"},{\"content\":{\"blockPath\":[],\"channel\":[111,1],\"dimensions\":[360,1],\"domain\":\"\",\"lineColor\":\"#7e2f8e\",\"lineWidth\":2,\"parentID\":1,\"port\":1,\"signalID\":112,\"signalName\":\"MATLAB Function1:1\"},\"type\":\"RecordBlkView.Signal\",\"uuid\":\"\"},{\"content\":{\"blockPath\":[],\"channel\":[112,1],\"dimensions\":[360,1],\"domain\":\"\",\"lineColor\":\"#77ac30\",\"lineWidth\":2,\"parentID\":1,\"port\":1,\"signalID\":113,\"signalName\":\"MATLAB Function1:1\"},\"type\":\"RecordBlkView.Signal\",\"uuid\":\"\"},{\"content\":{\"blockPath\":[],\"channel\":[113,1],\"dimensions\":[360,1],\"domain\":\"\",\"lineColor\":\"#4dbeee\",\"lineWidth\":2,\"parentID\":1,\"port\":1,\"signalID\":114,\"signalName\":\"MATLAB Function1:1\"},\"type\":\"RecordBlkView.Signal\",\"uuid\":\"\"},{\"content\":{\"blockPath\":[],\"channel\":[114,1],\"dimensions\":[360,1],\"domain\":\"\",\"lineColor\":\"#a2142f\",\"lineWidth\":2,\"parentID\":1,\"port\":1,\"signalID\":115,\"signalName\":\"MATLAB Function1:1\"},\"type\":\"RecordBlkView.Signal\",\"uuid\":\"\"},{\"content\":{\"blockPath\":[],\"channel\":[115,1],\"dimensions\":[360,1],\"domain\":\"\",\"lineColor\":\"#139fff\",\"lineWidth\":2,\"parentID\":1,\"port\":1,\"signalID\":116,\"signalName\":\"MATLAB Function1:1\"},\"type\":\"RecordBlkView.Signal\",\"uuid\":\"\"},{\"content\":{\"blockPath\":[],\"channel\":[116,1],\"dimensions\":[360,1],\"domain\":\"\",\"lineColor\":\"#ff6929\",\"lineWidth\":2,\"parentID\":1,\"port\":1,\"signalID\":117,\"signalName\":\"MATLAB Function1:1\"},\"type\":\"RecordBlkView.Signal\",\"uuid\":\"\"},{\"content\":{\"blockPath\":[],\"channel\":[117,1],\"dimensions\":[360,1],\"domain\":\"\",\"lineColor\":\"#b746ff\",\"lineWidth\":2,\"parentID\":1,\"port\":1,\"signalID\":118,\"signalName\":\"MATLAB Function1:1\"},\"type\":\"RecordBlkView.Signal\",\"uuid\":\"\"},{\"content\":{\"blockPath\":[],\"channel\":[118,1],\"dimensions\":[360,1],\"domain\":\"\",\"lineColor\":\"#64d413\",\"lineWidth\":2,\"parentID\":1,\"port\":1,\"signalID\":119,\"signalName\":\"MATLAB Function1:1\"},\"type\":\"RecordBlkView.Signal\",\"uuid\":\"\"},{\"content\":{\"blockPath\":[],\"channel\":[119,1],\"dimensions\":[360,1],\"domain\":\"\",\"lineColor\":\"#ff13a6\",\"lineWidth\":2,\"parentID\":1,\"port\":1,\"signalID\":120,\"signalName\":\"MATLAB Function1:1\"},\"type\":\"RecordBlkView.Signal\",\"uuid\":\"\"},{\"content\":{\"blockPath\":[],\"channel\":[120,1],\"dimensions\":[360,1],\"domain\":\"\",\"lineColor\":\"#fe330a\",\"lineWidth\":2,\"parentID\":1,\"port\":1,\"signalID\":121,\"signalName\":\"MATLAB Function1:1\"},\"type\":\"RecordBlkView.Signal\",\"uuid\":\"\"},{\"content\":{\"blockPath\":[],\"channel\":[121,1],\"dimensions\":[360,1],\"domain\":\"\",\"lineColor\":\"#22b573\",\"lineWidth\":2,\"parentID\":1,\"port\":1,\"signalID\":122,\"signalName\":\"MATLAB Function1:1\"},\"type\":\"RecordBlkView.Signal\",\"uuid\":\"\"},{\"content\":{\"blockPath\":[],\"channel\":[122,1],\"dimensions\":[360,1],\"domain\":\"\",\"lineColor\":\"#0072bd\",\"lineWidth\":2,\"parentID\":1,\"port\":1,\"signalID\":123,\"signalName\":\"MATLAB Function1:1\"},\"type\":\"RecordBlkView.Signal\",\"uuid\":\"\"},{\"content\":{\"blockPath\":[],\"channel\":[123,1],\"dimensions\":[360,1],\"domain\":\"\",\"lineColor\":\"#d95319\",\"lineWidth\":2,\"parentID\":1,\"port\":1,\"signalID\":124,\"signalName\":\"MATLAB Function1:1\"},\"type\":\"RecordBlkView.Signal\",\"uuid\":\"\"},{\"content\":{\"blockPath\":[],\"channel\":[124,1],\"dimensions\":[360,1],\"domain\":\"\",\"lineColor\":\"#edb120\",\"lineWidth\":2,\"parentID\":1,\"port\":1,\"signalID\":125,\"signalName\":\"MATLAB Function1:1\"},\"type\":\"RecordBlkView.Signal\",\"uuid\":\"\"},{\"content\":{\"blockPath\":[],\"channel\":[125,1],\"dimensions\":[360,1],\"domain\":\"\",\"lineColor\":\"#7e2f8e\",\"lineWidth\":2,\"parentID\":1,\"port\":1,\"signalID\":126,\"signalName\":\"MATLAB Function1:1\"},\"type\":\"RecordBlkView.Signal\",\"uuid\":\"\"},{\"content\":{\"blockPath\":[],\"channel\":[126,1],\"dimensions\":[360,1],\"domain\":\"\",\"lineColor\":\"#77ac30\",\"lineWidth\":2,\"parentID\":1,\"port\":1,\"signalID\":127,\"signalName\":\"MATLAB Function1:1\"},\"type\":\"RecordBlkView.Signal\",\"uuid\":\"\"},{\"content\":{\"blockPath\":[],\"channel\":[127,1],\"dimensions\":[360,1],\"domain\":\"\",\"lineColor\":\"#4dbeee\",\"lineWidth\":2,\"parentID\":1,\"port\":1,\"signalID\":128,\"signalName\":\"MATLAB Function1:1\"},\"type\":\"RecordBlkView.Signal\",\"uuid\":\"\"},{\"content\":{\"blockPath\":[],\"channel\":[128,1],\"dimensions\":[360,1],\"domain\":\"\",\"lineColor\":\"#a2142f\",\"lineWidth\":2,\"parentID\":1,\"port\":1,\"signalID\":129,\"signalName\":\"MATLAB Function1:1\"},\"type\":\"RecordBlkView.Signal\",\"uuid\":\"\"},{\"content\":{\"blockPath\":[],\"channel\":[129,1],\"dimensions\":[360,1],\"domain\":\"\",\"lineColor\":\"#139fff\",\"lineWidth\":2,\"parentID\":1,\"port\":1,\"signalID\":130,\"signalName\":\"MATLAB Function1:1\"},\"type\":\"RecordBlkView.Signal\",\"uuid\":\"\"},{\"content\":{\"blockPath\":[],\"channel\":[130,1],\"dimensions\":[360,1],\"domain\":\"\",\"lineColor\":\"#ff6929\",\"lineWidth\":2,\"parentID\":1,\"port\":1,\"signalID\":131,\"signalName\":\"MATLAB Function1:1\"},\"type\":\"RecordBlkView.Signal\",\"uuid\":\"\"},{\"content\":{\"blockPath\":[],\"channel\":[131,1],\"dimensions\":[360,1],\"domain\":\"\",\"lineColor\":\"#b746ff\",\"lineWidth\":2,\"parentID\":1,\"port\":1,\"signalID\":132,\"signalName\":\"MATLAB Function1:1\"},\"type\":\"RecordBlkView.Signal\",\"uuid\":\"\"},{\"content\":{\"blockPath\":[],\"channel\":[132,1],\"dimensions\":[360,1],\"domain\":\"\",\"lineColor\":\"#64d413\",\"lineWidth\":2,\"parentID\":1,\"port\":1,\"signalID\":133,\"signalName\":\"MATLAB Function1:1\"},\"type\":\"RecordBlkView.Signal\",\"uuid\":\"\"},{\"content\":{\"blockPath\":[],\"channel\":[133,1],\"dimensions\":[360,1],\"domain\":\"\",\"lineColor\":\"#ff13a6\",\"lineWidth\":2,\"parentID\":1,\"port\":1,\"signalID\":134,\"signalName\":\"MATLAB Function1:1\"},\"type\":\"RecordBlkView.Signal\",\"uuid\":\"\"},{\"content\":{\"blockPath\":[],\"channel\":[134,1],\"dimensions\":[360,1],\"domain\":\"\",\"lineColor\":\"#fe330a\",\"lineWidth\":2,\"parentID\":1,\"port\":1,\"signalID\":135,\"signalName\":\"MATLAB Function1:1\"},\"type\":\"RecordBlkView.Signal\",\"uuid\":\"\"},{\"content\":{\"blockPath\":[],\"channel\":[135,1],\"dimensions\":[360,1],\"domain\":\"\",\"lineColor\":\"#22b573\",\"lineWidth\":2,\"parentID\":1,\"port\":1,\"signalID\":136,\"signalName\":\"MATLAB Function1:1\"},\"type\":\"RecordBlkView.Signal\",\"uuid\":\"\"},{\"content\":{\"blockPath\":[],\"channel\":[136,1],\"dimensions\":[360,1],\"domain\":\"\",\"lineColor\":\"#0072bd\",\"lineWidth\":2,\"parentID\":1,\"port\":1,\"signalID\":137,\"signalName\":\"MATLAB Function1:1\"},\"type\":\"RecordBlkView.Signal\",\"uuid\":\"\"},{\"content\":{\"blockPath\":[],\"channel\":[137,1],\"dimensions\":[360,1],\"domain\":\"\",\"lineColor\":\"#d95319\",\"lineWidth\":2,\"parentID\":1,\"port\":1,\"signalID\":138,\"signalName\":\"MATLAB Function1:1\"},\"type\":\"RecordBlkView.Signal\",\"uuid\":\"\"},{\"content\":{\"blockPath\":[],\"channel\":[138,1],\"dimensions\":[360,1],\"domain\":\"\",\"lineColor\":\"#edb120\",\"lineWidth\":2,\"parentID\":1,\"port\":1,\"signalID\":139,\"signalName\":\"MATLAB Function1:1\"},\"type\":\"RecordBlkView.Signal\",\"uuid\":\"\"},{\"content\":{\"blockPath\":[],\"channel\":[139,1],\"dimensions\":[360,1],\"domain\":\"\",\"lineColor\":\"#7e2f8e\",\"lineWidth\":2,\"parentID\":1,\"port\":1,\"signalID\":140,\"signalName\":\"MATLAB Function1:1\"},\"type\":\"RecordBlkView.Signal\",\"uuid\":\"\"},{\"content\":{\"blockPath\":[],\"channel\":[140,1],\"dimensions\":[360,1],\"domain\":\"\",\"lineColor\":\"#77ac30\",\"lineWidth\":2,\"parentID\":1,\"port\":1,\"signalID\":141,\"signalName\":\"MATLAB Function1:1\"},\"type\":\"RecordBlkView.Signal\",\"uuid\":\"\"},{\"content\":{\"blockPath\":[],\"channel\":[141,1],\"dimensions\":[360,1],\"domain\":\"\",\"lineColor\":\"#4dbeee\",\"lineWidth\":2,\"parentID\":1,\"port\":1,\"signalID\":142,\"signalName\":\"MATLAB Function1:1\"},\"type\":\"RecordBlkView.Signal\",\"uuid\":\"\"},{\"content\":{\"blockPath\":[],\"channel\":[142,1],\"dimensions\":[360,1],\"domain\":\"\",\"lineColor\":\"#a2142f\",\"lineWidth\":2,\"parentID\":1,\"port\":1,\"signalID\":143,\"signalName\":\"MATLAB Function1:1\"},\"type\":\"RecordBlkView.Signal\",\"uuid\":\"\"},{\"content\":{\"blockPath\":[],\"channel\":[143,1],\"dimensions\":[360,1],\"domain\":\"\",\"lineColor\":\"#139fff\",\"lineWidth\":2,\"parentID\":1,\"port\":1,\"signalID\":144,\"signalName\":\"MATLAB Function1:1\"},\"type\":\"RecordBlkView.Signal\",\"uuid\":\"\"},{\"content\":{\"blockPath\":[],\"channel\":[144,1],\"dimensions\":[360,1],\"domain\":\"\",\"lineColor\":\"#ff6929\",\"lineWidth\":2,\"parentID\":1,\"port\":1,\"signalID\":145,\"signalName\":\"MATLAB Function1:1\"},\"type\":\"RecordBlkView.Signal\",\"uuid\":\"\"},{\"content\":{\"blockPath\":[],\"channel\":[145,1],\"dimensions\":[360,1],\"domain\":\"\",\"lineColor\":\"#b746ff\",\"lineWidth\":2,\"parentID\":1,\"port\":1,\"signalID\":146,\"signalName\":\"MATLAB Function1:1\"},\"type\":\"RecordBlkView.Signal\",\"uuid\":\"\"},{\"content\":{\"blockPath\":[],\"channel\":[146,1],\"dimensions\":[360,1],\"domain\":\"\",\"lineColor\":\"#64d413\",\"lineWidth\":2,\"parentID\":1,\"port\":1,\"signalID\":147,\"signalName\":\"MATLAB Function1:1\"},\"type\":\"RecordBlkView.Signal\",\"uuid\":\"\"},{\"content\":{\"blockPath\":[],\"channel\":[147,1],\"dimensions\":[360,1],\"domain\":\"\",\"lineColor\":\"#ff13a6\",\"lineWidth\":2,\"parentID\":1,\"port\":1,\"signalID\":148,\"signalName\":\"MATLAB Function1:1\"},\"type\":\"RecordBlkView.Signal\",\"uuid\":\"\"},{\"content\":{\"blockPath\":[],\"channel\":[148,1],\"dimensions\":[360,1],\"domain\":\"\",\"lineColor\":\"#fe330a\",\"lineWidth\":2,\"parentID\":1,\"port\":1,\"signalID\":149,\"signalName\":\"MATLAB Function1:1\"},\"type\":\"RecordBlkView.Signal\",\"uuid\":\"\"},{\"content\":{\"blockPath\":[],\"channel\":[149,1],\"dimensions\":[360,1],\"domain\":\"\",\"lineColor\":\"#22b573\",\"lineWidth\":2,\"parentID\":1,\"port\":1,\"signalID\":150,\"signalName\":\"MATLAB Function1:1\"},\"type\":\"RecordBlkView.Signal\",\"uuid\":\"\"},{\"content\":{\"blockPath\":[],\"channel\":[150,1],\"dimensions\":[360,1],\"domain\":\"\",\"lineColor\":\"#0072bd\",\"lineWidth\":2,\"parentID\":1,\"port\":1,\"signalID\":151,\"signalName\":\"MATLAB Function1:1\"},\"type\":\"RecordBlkView.Signal\",\"uuid\":\"\"},{\"content\":{\"blockPath\":[],\"channel\":[151,1],\"dimensions\":[360,1],\"domain\":\"\",\"lineColor\":\"#d95319\",\"lineWidth\":2,\"parentID\":1,\"port\":1,\"signalID\":152,\"signalName\":\"MATLAB Function1:1\"},\"type\":\"RecordBlkView.Signal\",\"uuid\":\"\"},{\"content\":{\"blockPath\":[],\"channel\":[152,1],\"dimensions\":[360,1],\"domain\":\"\",\"lineColor\":\"#edb120\",\"lineWidth\":2,\"parentID\":1,\"port\":1,\"signalID\":153,\"signalName\":\"MATLAB Function1:1\"},\"type\":\"RecordBlkView.Signal\",\"uuid\":\"\"},{\"content\":{\"blockPath\":[],\"channel\":[153,1],\"dimensions\":[360,1],\"domain\":\"\",\"lineColor\":\"#7e2f8e\",\"lineWidth\":2,\"parentID\":1,\"port\":1,\"signalID\":154,\"signalName\":\"MATLAB Function1:1\"},\"type\":\"RecordBlkView.Signal\",\"uuid\":\"\"},{\"content\":{\"blockPath\":[],\"channel\":[154,1],\"dimensions\":[360,1],\"domain\":\"\",\"lineColor\":\"#77ac30\",\"lineWidth\":2,\"parentID\":1,\"port\":1,\"signalID\":155,\"signalName\":\"MATLAB Function1:1\"},\"type\":\"RecordBlkView.Signal\",\"uuid\":\"\"},{\"content\":{\"blockPath\":[],\"channel\":[155,1],\"dimensions\":[360,1],\"domain\":\"\",\"lineColor\":\"#4dbeee\",\"lineWidth\":2,\"parentID\":1,\"port\":1,\"signalID\":156,\"signalName\":\"MATLAB Function1:1\"},\"type\":\"RecordBlkView.Signal\",\"uuid\":\"\"},{\"content\":{\"blockPath\":[],\"channel\":[156,1],\"dimensions\":[360,1],\"domain\":\"\",\"lineColor\":\"#a2142f\",\"lineWidth\":2,\"parentID\":1,\"port\":1,\"signalID\":157,\"signalName\":\"MATLAB Function1:1\"},\"type\":\"RecordBlkView.Signal\",\"uuid\":\"\"},{\"content\":{\"blockPath\":[],\"channel\":[157,1],\"dimensions\":[360,1],\"domain\":\"\",\"lineColor\":\"#139fff\",\"lineWidth\":2,\"parentID\":1,\"port\":1,\"signalID\":158,\"signalName\":\"MATLAB Function1:1\"},\"type\":\"RecordBlkView.Signal\",\"uuid\":\"\"},{\"content\":{\"blockPath\":[],\"channel\":[158,1],\"dimensions\":[360,1],\"domain\":\"\",\"lineColor\":\"#ff6929\",\"lineWidth\":2,\"parentID\":1,\"port\":1,\"signalID\":159,\"signalName\":\"MATLAB Function1:1\"},\"type\":\"RecordBlkView.Signal\",\"uuid\":\"\"},{\"content\":{\"blockPath\":[],\"channel\":[159,1],\"dimensions\":[360,1],\"domain\":\"\",\"lineColor\":\"#b746ff\",\"lineWidth\":2,\"parentID\":1,\"port\":1,\"signalID\":160,\"signalName\":\"MATLAB Function1:1\"},\"type\":\"RecordBlkView.Signal\",\"uuid\":\"\"},{\"content\":{\"blockPath\":[],\"channel\":[160,1],\"dimensions\":[360,1],\"domain\":\"\",\"lineColor\":\"#64d413\",\"lineWidth\":2,\"parentID\":1,\"port\":1,\"signalID\":161,\"signalName\":\"MATLAB Function1:1\"},\"type\":\"RecordBlkView.Signal\",\"uuid\":\"\"},{\"content\":{\"blockPath\":[],\"channel\":[161,1],\"dimensions\":[360,1],\"domain\":\"\",\"lineColor\":\"#ff13a6\",\"lineWidth\":2,\"parentID\":1,\"port\":1,\"signalID\":162,\"signalName\":\"MATLAB Function1:1\"},\"type\":\"RecordBlkView.Signal\",\"uuid\":\"\"},{\"content\":{\"blockPath\":[],\"channel\":[162,1],\"dimensions\":[360,1],\"domain\":\"\",\"lineColor\":\"#fe330a\",\"lineWidth\":2,\"parentID\":1,\"port\":1,\"signalID\":163,\"signalName\":\"MATLAB Function1:1\"},\"type\":\"RecordBlkView.Signal\",\"uuid\":\"\"},{\"content\":{\"blockPath\":[],\"channel\":[163,1],\"dimensions\":[360,1],\"domain\":\"\",\"lineColor\":\"#22b573\",\"lineWidth\":2,\"parentID\":1,\"port\":1,\"signalID\":164,\"signalName\":\"MATLAB Function1:1\"},\"type\":\"RecordBlkView.Signal\",\"uuid\":\"\"},{\"content\":{\"blockPath\":[],\"channel\":[164,1],\"dimensions\":[360,1],\"domain\":\"\",\"lineColor\":\"#0072bd\",\"lineWidth\":2,\"parentID\":1,\"port\":1,\"signalID\":165,\"signalName\":\"MATLAB Function1:1\"},\"type\":\"RecordBlkView.Signal\",\"uuid\":\"\"},{\"content\":{\"blockPath\":[],\"channel\":[165,1],\"dimensions\":[360,1],\"domain\":\"\",\"lineColor\":\"#d95319\",\"lineWidth\":2,\"parentID\":1,\"port\":1,\"signalID\":166,\"signalName\":\"MATLAB Function1:1\"},\"type\":\"RecordBlkView.Signal\",\"uuid\":\"\"},{\"content\":{\"blockPath\":[],\"channel\":[166,1],\"dimensions\":[360,1],\"domain\":\"\",\"lineColor\":\"#edb120\",\"lineWidth\":2,\"parentID\":1,\"port\":1,\"signalID\":167,\"signalName\":\"MATLAB Function1:1\"},\"type\":\"RecordBlkView.Signal\",\"uuid\":\"\"},{\"content\":{\"blockPath\":[],\"channel\":[167,1],\"dimensions\":[360,1],\"domain\":\"\",\"lineColor\":\"#7e2f8e\",\"lineWidth\":2,\"parentID\":1,\"port\":1,\"signalID\":168,\"signalName\":\"MATLAB Function1:1\"},\"type\":\"RecordBlkView.Signal\",\"uuid\":\"\"},{\"content\":{\"blockPath\":[],\"channel\":[168,1],\"dimensions\":[360,1],\"domain\":\"\",\"lineColor\":\"#77ac30\",\"lineWidth\":2,\"parentID\":1,\"port\":1,\"signalID\":169,\"signalName\":\"MATLAB Function1:1\"},\"type\":\"RecordBlkView.Signal\",\"uuid\":\"\"},{\"content\":{\"blockPath\":[],\"channel\":[169,1],\"dimensions\":[360,1],\"domain\":\"\",\"lineColor\":\"#4dbeee\",\"lineWidth\":2,\"parentID\":1,\"port\":1,\"signalID\":170,\"signalName\":\"MATLAB Function1:1\"},\"type\":\"RecordBlkView.Signal\",\"uuid\":\"\"},{\"content\":{\"blockPath\":[],\"channel\":[170,1],\"dimensions\":[360,1],\"domain\":\"\",\"lineColor\":\"#a2142f\",\"lineWidth\":2,\"parentID\":1,\"port\":1,\"signalID\":171,\"signalName\":\"MATLAB Function1:1\"},\"type\":\"RecordBlkView.Signal\",\"uuid\":\"\"},{\"content\":{\"blockPath\":[],\"channel\":[171,1],\"dimensions\":[360,1],\"domain\":\"\",\"lineColor\":\"#139fff\",\"lineWidth\":2,\"parentID\":1,\"port\":1,\"signalID\":172,\"signalName\":\"MATLAB Function1:1\"},\"type\":\"RecordBlkView.Signal\",\"uuid\":\"\"},{\"content\":{\"blockPath\":[],\"channel\":[172,1],\"dimensions\":[360,1],\"domain\":\"\",\"lineColor\":\"#ff6929\",\"lineWidth\":2,\"parentID\":1,\"port\":1,\"signalID\":173,\"signalName\":\"MATLAB Function1:1\"},\"type\":\"RecordBlkView.Signal\",\"uuid\":\"\"},{\"content\":{\"blockPath\":[],\"channel\":[173,1],\"dimensions\":[360,1],\"domain\":\"\",\"lineColor\":\"#b746ff\",\"lineWidth\":2,\"parentID\":1,\"port\":1,\"signalID\":174,\"signalName\":\"MATLAB Function1:1\"},\"type\":\"RecordBlkView.Signal\",\"uuid\":\"\"},{\"content\":{\"blockPath\":[],\"channel\":[174,1],\"dimensions\":[360,1],\"domain\":\"\",\"lineColor\":\"#64d413\",\"lineWidth\":2,\"parentID\":1,\"port\":1,\"signalID\":175,\"signalName\":\"MATLAB Function1:1\"},\"type\":\"RecordBlkView.Signal\",\"uuid\":\"\"},{\"content\":{\"blockPath\":[],\"channel\":[175,1],\"dimensions\":[360,1],\"domain\":\"\",\"lineColor\":\"#ff13a6\",\"lineWidth\":2,\"parentID\":1,\"port\":1,\"signalID\":176,\"signalName\":\"MATLAB Function1:1\"},\"type\":\"RecordBlkView.Signal\",\"uuid\":\"\"},{\"content\":{\"blockPath\":[],\"channel\":[176,1],\"dimensions\":[360,1],\"domain\":\"\",\"lineColor\":\"#fe330a\",\"lineWidth\":2,\"parentID\":1,\"port\":1,\"signalID\":177,\"signalName\":\"MATLAB Function1:1\"},\"type\":\"RecordBlkView.Signal\",\"uuid\":\"\"},{\"content\":{\"blockPath\":[],\"channel\":[177,1],\"dimensions\":[360,1],\"domain\":\"\",\"lineColor\":\"#22b573\",\"lineWidth\":2,\"parentID\":1,\"port\":1,\"signalID\":178,\"signalName\":\"MATLAB Function1:1\"},\"type\":\"RecordBlkView.Signal\",\"uuid\":\"\"},{\"content\":{\"blockPath\":[],\"channel\":[178,1],\"dimensions\":[360,1],\"domain\":\"\",\"lineColor\":\"#0072bd\",\"lineWidth\":2,\"parentID\":1,\"port\":1,\"signalID\":179,\"signalName\":\"MATLAB Function1:1\"},\"type\":\"RecordBlkView.Signal\",\"uuid\":\"\"},{\"content\":{\"blockPath\":[],\"channel\":[179,1],\"dimensions\":[360,1],\"domain\":\"\",\"lineColor\":\"#d95319\",\"lineWidth\":2,\"parentID\":1,\"port\":1,\"signalID\":180,\"signalName\":\"MATLAB Function1:1\"},\"type\":\"RecordBlkView.Signal\",\"uuid\":\"\"},{\"content\":{\"blockPath\":[],\"channel\":[180,1],\"dimensions\":[360,1],\"domain\":\"\",\"lineColor\":\"#edb120\",\"lineWidth\":2,\"parentID\":1,\"port\":1,\"signalID\":181,\"signalName\":\"MATLAB Function1:1\"},\"type\":\"RecordBlkView.Signal\",\"uuid\":\"\"},{\"content\":{\"blockPath\":[],\"channel\":[181,1],\"dimensions\":[360,1],\"domain\":\"\",\"lineColor\":\"#7e2f8e\",\"lineWidth\":2,\"parentID\":1,\"port\":1,\"signalID\":182,\"signalName\":\"MATLAB Function1:1\"},\"type\":\"RecordBlkView.Signal\",\"uuid\":\"\"},{\"content\":{\"blockPath\":[],\"channel\":[182,1],\"dimensions\":[360,1],\"domain\":\"\",\"lineColor\":\"#77ac30\",\"lineWidth\":2,\"parentID\":1,\"port\":1,\"signalID\":183,\"signalName\":\"MATLAB Function1:1\"},\"type\":\"RecordBlkView.Signal\",\"uuid\":\"\"},{\"content\":{\"blockPath\":[],\"channel\":[183,1],\"dimensions\":[360,1],\"domain\":\"\",\"lineColor\":\"#4dbeee\",\"lineWidth\":2,\"parentID\":1,\"port\":1,\"signalID\":184,\"signalName\":\"MATLAB Function1:1\"},\"type\":\"RecordBlkView.Signal\",\"uuid\":\"\"},{\"content\":{\"blockPath\":[],\"channel\":[184,1],\"dimensions\":[360,1],\"domain\":\"\",\"lineColor\":\"#a2142f\",\"lineWidth\":2,\"parentID\":1,\"port\":1,\"signalID\":185,\"signalName\":\"MATLAB Function1:1\"},\"type\":\"RecordBlkView.Signal\",\"uuid\":\"\"},{\"content\":{\"blockPath\":[],\"channel\":[185,1],\"dimensions\":[360,1],\"domain\":\"\",\"lineColor\":\"#139fff\",\"lineWidth\":2,\"parentID\":1,\"port\":1,\"signalID\":186,\"signalName\":\"MATLAB Function1:1\"},\"type\":\"RecordBlkView.Signal\",\"uuid\":\"\"},{\"content\":{\"blockPath\":[],\"channel\":[186,1],\"dimensions\":[360,1],\"domain\":\"\",\"lineColor\":\"#ff6929\",\"lineWidth\":2,\"parentID\":1,\"port\":1,\"signalID\":187,\"signalName\":\"MATLAB Function1:1\"},\"type\":\"RecordBlkView.Signal\",\"uuid\":\"\"},{\"content\":{\"blockPath\":[],\"channel\":[187,1],\"dimensions\":[360,1],\"domain\":\"\",\"lineColor\":\"#b746ff\",\"lineWidth\":2,\"parentID\":1,\"port\":1,\"signalID\":188,\"signalName\":\"MATLAB Function1:1\"},\"type\":\"RecordBlkView.Signal\",\"uuid\":\"\"},{\"content\":{\"blockPath\":[],\"channel\":[188,1],\"dimensions\":[360,1],\"domain\":\"\",\"lineColor\":\"#64d413\",\"lineWidth\":2,\"parentID\":1,\"port\":1,\"signalID\":189,\"signalName\":\"MATLAB Function1:1\"},\"type\":\"RecordBlkView.Signal\",\"uuid\":\"\"},{\"content\":{\"blockPath\":[],\"channel\":[189,1],\"dimensions\":[360,1],\"domain\":\"\",\"lineColor\":\"#ff13a6\",\"lineWidth\":2,\"parentID\":1,\"port\":1,\"signalID\":190,\"signalName\":\"MATLAB Function1:1\"},\"type\":\"RecordBlkView.Signal\",\"uuid\":\"\"},{\"content\":{\"blockPath\":[],\"channel\":[190,1],\"dimensions\":[360,1],\"domain\":\"\",\"lineColor\":\"#fe330a\",\"lineWidth\":2,\"parentID\":1,\"port\":1,\"signalID\":191,\"signalName\":\"MATLAB Function1:1\"},\"type\":\"RecordBlkView.Signal\",\"uuid\":\"\"},{\"content\":{\"blockPath\":[],\"channel\":[191,1],\"dimensions\":[360,1],\"domain\":\"\",\"lineColor\":\"#22b573\",\"lineWidth\":2,\"parentID\":1,\"port\":1,\"signalID\":192,\"signalName\":\"MATLAB Function1:1\"},\"type\":\"RecordBlkView.Signal\",\"uuid\":\"\"},{\"content\":{\"blockPath\":[],\"channel\":[192,1],\"dimensions\":[360,1],\"domain\":\"\",\"lineColor\":\"#0072bd\",\"lineWidth\":2,\"parentID\":1,\"port\":1,\"signalID\":193,\"signalName\":\"MATLAB Function1:1\"},\"type\":\"RecordBlkView.Signal\",\"uuid\":\"\"},{\"content\":{\"blockPath\":[],\"channel\":[193,1],\"dimensions\":[360,1],\"domain\":\"\",\"lineColor\":\"#d95319\",\"lineWidth\":2,\"parentID\":1,\"port\":1,\"signalID\":194,\"signalName\":\"MATLAB Function1:1\"},\"type\":\"RecordBlkView.Signal\",\"uuid\":\"\"},{\"content\":{\"blockPath\":[],\"channel\":[194,1],\"dimensions\":[360,1],\"domain\":\"\",\"lineColor\":\"#edb120\",\"lineWidth\":2,\"parentID\":1,\"port\":1,\"signalID\":195,\"signalName\":\"MATLAB Function1:1\"},\"type\":\"RecordBlkView.Signal\",\"uuid\":\"\"},{\"content\":{\"blockPath\":[],\"channel\":[195,1],\"dimensions\":[360,1],\"domain\":\"\",\"lineColor\":\"#7e2f8e\",\"lineWidth\":2,\"parentID\":1,\"port\":1,\"signalID\":196,\"signalName\":\"MATLAB Function1:1\"},\"type\":\"RecordBlkView.Signal\",\"uuid\":\"\"},{\"content\":{\"blockPath\":[],\"channel\":[196,1],\"dimensions\":[360,1],\"domain\":\"\",\"lineColor\":\"#77ac30\",\"lineWidth\":2,\"parentID\":1,\"port\":1,\"signalID\":197,\"signalName\":\"MATLAB Function1:1\"},\"type\":\"RecordBlkView.Signal\",\"uuid\":\"\"},{\"content\":{\"blockPath\":[],\"channel\":[197,1],\"dimensions\":[360,1],\"domain\":\"\",\"lineColor\":\"#4dbeee\",\"lineWidth\":2,\"parentID\":1,\"port\":1,\"signalID\":198,\"signalName\":\"MATLAB Function1:1\"},\"type\":\"RecordBlkView.Signal\",\"uuid\":\"\"},{\"content\":{\"blockPath\":[],\"channel\":[198,1],\"dimensions\":[360,1],\"domain\":\"\",\"lineColor\":\"#a2142f\",\"lineWidth\":2,\"parentID\":1,\"port\":1,\"signalID\":199,\"signalName\":\"MATLAB Function1:1\"},\"type\":\"RecordBlkView.Signal\",\"uuid\":\"\"},{\"content\":{\"blockPath\":[],\"channel\":[199,1],\"dimensions\":[360,1],\"domain\":\"\",\"lineColor\":\"#139fff\",\"lineWidth\":2,\"parentID\":1,\"port\":1,\"signalID\":200,\"signalName\":\"MATLAB Function1:1\"},\"type\":\"RecordBlkView.Signal\",\"uuid\":\"\"},{\"content\":{\"blockPath\":[],\"channel\":[200,1],\"dimensions\":[360,1],\"domain\":\"\",\"lineColor\":\"#ff6929\",\"lineWidth\":2,\"parentID\":1,\"port\":1,\"signalID\":201,\"signalName\":\"MATLAB Function1:1\"},\"type\":\"RecordBlkView.Signal\",\"uuid\":\"\"},{\"content\":{\"blockPath\":[],\"channel\":[201,1],\"dimensions\":[360,1],\"domain\":\"\",\"lineColor\":\"#b746ff\",\"lineWidth\":2,\"parentID\":1,\"port\":1,\"signalID\":202,\"signalName\":\"MATLAB Function1:1\"},\"type\":\"RecordBlkView.Signal\",\"uuid\":\"\"},{\"content\":{\"blockPath\":[],\"channel\":[202,1],\"dimensions\":[360,1],\"domain\":\"\",\"lineColor\":\"#64d413\",\"lineWidth\":2,\"parentID\":1,\"port\":1,\"signalID\":203,\"signalName\":\"MATLAB Function1:1\"},\"type\":\"RecordBlkView.Signal\",\"uuid\":\"\"},{\"content\":{\"blockPath\":[],\"channel\":[203,1],\"dimensions\":[360,1],\"domain\":\"\",\"lineColor\":\"#ff13a6\",\"lineWidth\":2,\"parentID\":1,\"port\":1,\"signalID\":204,\"signalName\":\"MATLAB Function1:1\"},\"type\":\"RecordBlkView.Signal\",\"uuid\":\"\"},{\"content\":{\"blockPath\":[],\"channel\":[204,1],\"dimensions\":[360,1],\"domain\":\"\",\"lineColor\":\"#fe330a\",\"lineWidth\":2,\"parentID\":1,\"port\":1,\"signalID\":205,\"signalName\":\"MATLAB Function1:1\"},\"type\":\"RecordBlkView.Signal\",\"uuid\":\"\"},{\"content\":{\"blockPath\":[],\"channel\":[205,1],\"dimensions\":[360,1],\"domain\":\"\",\"lineColor\":\"#22b573\",\"lineWidth\":2,\"parentID\":1,\"port\":1,\"signalID\":206,\"signalName\":\"MATLAB Function1:1\"},\"type\":\"RecordBlkView.Signal\",\"uuid\":\"\"},{\"content\":{\"blockPath\":[],\"channel\":[206,1],\"dimensions\":[360,1],\"domain\":\"\",\"lineColor\":\"#0072bd\",\"lineWidth\":2,\"parentID\":1,\"port\":1,\"signalID\":207,\"signalName\":\"MATLAB Function1:1\"},\"type\":\"RecordBlkView.Signal\",\"uuid\":\"\"},{\"content\":{\"blockPath\":[],\"channel\":[207,1],\"dimensions\":[360,1],\"domain\":\"\",\"lineColor\":\"#d95319\",\"lineWidth\":2,\"parentID\":1,\"port\":1,\"signalID\":208,\"signalName\":\"MATLAB Function1:1\"},\"type\":\"RecordBlkView.Signal\",\"uuid\":\"\"},{\"content\":{\"blockPath\":[],\"channel\":[208,1],\"dimensions\":[360,1],\"domain\":\"\",\"lineColor\":\"#edb120\",\"lineWidth\":2,\"parentID\":1,\"port\":1,\"signalID\":209,\"signalName\":\"MATLAB Function1:1\"},\"type\":\"RecordBlkView.Signal\",\"uuid\":\"\"},{\"content\":{\"blockPath\":[],\"channel\":[209,1],\"dimensions\":[360,1],\"domain\":\"\",\"lineColor\":\"#7e2f8e\",\"lineWidth\":2,\"parentID\":1,\"port\":1,\"signalID\":210,\"signalName\":\"MATLAB Function1:1\"},\"type\":\"RecordBlkView.Signal\",\"uuid\":\"\"},{\"content\":{\"blockPath\":[],\"channel\":[210,1],\"dimensions\":[360,1],\"domain\":\"\",\"lineColor\":\"#77ac30\",\"lineWidth\":2,\"parentID\":1,\"port\":1,\"signalID\":211,\"signalName\":\"MATLAB Function1:1\"},\"type\":\"RecordBlkView.Signal\",\"uuid\":\"\"},{\"content\":{\"blockPath\":[],\"channel\":[211,1],\"dimensions\":[360,1],\"domain\":\"\",\"lineColor\":\"#4dbeee\",\"lineWidth\":2,\"parentID\":1,\"port\":1,\"signalID\":212,\"signalName\":\"MATLAB Function1:1\"},\"type\":\"RecordBlkView.Signal\",\"uuid\":\"\"},{\"content\":{\"blockPath\":[],\"channel\":[212,1],\"dimensions\":[360,1],\"domain\":\"\",\"lineColor\":\"#a2142f\",\"lineWidth\":2,\"parentID\":1,\"port\":1,\"signalID\":213,\"signalName\":\"MATLAB Function1:1\"},\"type\":\"RecordBlkView.Signal\",\"uuid\":\"\"},{\"content\":{\"blockPath\":[],\"channel\":[213,1],\"dimensions\":[360,1],\"domain\":\"\",\"lineColor\":\"#139fff\",\"lineWidth\":2,\"parentID\":1,\"port\":1,\"signalID\":214,\"signalName\":\"MATLAB Function1:1\"},\"type\":\"RecordBlkView.Signal\",\"uuid\":\"\"},{\"content\":{\"blockPath\":[],\"channel\":[214,1],\"dimensions\":[360,1],\"domain\":\"\",\"lineColor\":\"#ff6929\",\"lineWidth\":2,\"parentID\":1,\"port\":1,\"signalID\":215,\"signalName\":\"MATLAB Function1:1\"},\"type\":\"RecordBlkView.Signal\",\"uuid\":\"\"},{\"content\":{\"blockPath\":[],\"channel\":[215,1],\"dimensions\":[360,1],\"domain\":\"\",\"lineColor\":\"#b746ff\",\"lineWidth\":2,\"parentID\":1,\"port\":1,\"signalID\":216,\"signalName\":\"MATLAB Function1:1\"},\"type\":\"RecordBlkView.Signal\",\"uuid\":\"\"},{\"content\":{\"blockPath\":[],\"channel\":[216,1],\"dimensions\":[360,1],\"domain\":\"\",\"lineColor\":\"#64d413\",\"lineWidth\":2,\"parentID\":1,\"port\":1,\"signalID\":217,\"signalName\":\"MATLAB Function1:1\"},\"type\":\"RecordBlkView.Signal\",\"uuid\":\"\"},{\"content\":{\"blockPath\":[],\"channel\":[217,1],\"dimensions\":[360,1],\"domain\":\"\",\"lineColor\":\"#ff13a6\",\"lineWidth\":2,\"parentID\":1,\"port\":1,\"signalID\":218,\"signalName\":\"MATLAB Function1:1\"},\"type\":\"RecordBlkView.Signal\",\"uuid\":\"\"},{\"content\":{\"blockPath\":[],\"channel\":[218,1],\"dimensions\":[360,1],\"domain\":\"\",\"lineColor\":\"#fe330a\",\"lineWidth\":2,\"parentID\":1,\"port\":1,\"signalID\":219,\"signalName\":\"MATLAB Function1:1\"},\"type\":\"RecordBlkView.Signal\",\"uuid\":\"\"},{\"content\":{\"blockPath\":[],\"channel\":[219,1],\"dimensions\":[360,1],\"domain\":\"\",\"lineColor\":\"#22b573\",\"lineWidth\":2,\"parentID\":1,\"port\":1,\"signalID\":220,\"signalName\":\"MATLAB Function1:1\"},\"type\":\"RecordBlkView.Signal\",\"uuid\":\"\"},{\"content\":{\"blockPath\":[],\"channel\":[220,1],\"dimensions\":[360,1],\"domain\":\"\",\"lineColor\":\"#0072bd\",\"lineWidth\":2,\"parentID\":1,\"port\":1,\"signalID\":221,\"signalName\":\"MATLAB Function1:1\"},\"type\":\"RecordBlkView.Signal\",\"uuid\":\"\"},{\"content\":{\"blockPath\":[],\"channel\":[221,1],\"dimensions\":[360,1],\"domain\":\"\",\"lineColor\":\"#d95319\",\"lineWidth\":2,\"parentID\":1,\"port\":1,\"signalID\":222,\"signalName\":\"MATLAB Function1:1\"},\"type\":\"RecordBlkView.Signal\",\"uuid\":\"\"},{\"content\":{\"blockPath\":[],\"channel\":[222,1],\"dimensions\":[360,1],\"domain\":\"\",\"lineColor\":\"#edb120\",\"lineWidth\":2,\"parentID\":1,\"port\":1,\"signalID\":223,\"signalName\":\"MATLAB Function1:1\"},\"type\":\"RecordBlkView.Signal\",\"uuid\":\"\"},{\"content\":{\"blockPath\":[],\"channel\":[223,1],\"dimensions\":[360,1],\"domain\":\"\",\"lineColor\":\"#7e2f8e\",\"lineWidth\":2,\"parentID\":1,\"port\":1,\"signalID\":224,\"signalName\":\"MATLAB Function1:1\"},\"type\":\"RecordBlkView.Signal\",\"uuid\":\"\"},{\"content\":{\"blockPath\":[],\"channel\":[224,1],\"dimensions\":[360,1],\"domain\":\"\",\"lineColor\":\"#77ac30\",\"lineWidth\":2,\"parentID\":1,\"port\":1,\"signalID\":225,\"signalName\":\"MATLAB Function1:1\"},\"type\":\"RecordBlkView.Signal\",\"uuid\":\"\"},{\"content\":{\"blockPath\":[],\"channel\":[225,1],\"dimensions\":[360,1],\"domain\":\"\",\"lineColor\":\"#4dbeee\",\"lineWidth\":2,\"parentID\":1,\"port\":1,\"signalID\":226,\"signalName\":\"MATLAB Function1:1\"},\"type\":\"RecordBlkView.Signal\",\"uuid\":\"\"},{\"content\":{\"blockPath\":[],\"channel\":[226,1],\"dimensions\":[360,1],\"domain\":\"\",\"lineColor\":\"#a2142f\",\"lineWidth\":2,\"parentID\":1,\"port\":1,\"signalID\":227,\"signalName\":\"MATLAB Function1:1\"},\"type\":\"RecordBlkView.Signal\",\"uuid\":\"\"},{\"content\":{\"blockPath\":[],\"channel\":[227,1],\"dimensions\":[360,1],\"domain\":\"\",\"lineColor\":\"#139fff\",\"lineWidth\":2,\"parentID\":1,\"port\":1,\"signalID\":228,\"signalName\":\"MATLAB Function1:1\"},\"type\":\"RecordBlkView.Signal\",\"uuid\":\"\"},{\"content\":{\"blockPath\":[],\"channel\":[228,1],\"dimensions\":[360,1],\"domain\":\"\",\"lineColor\":\"#ff6929\",\"lineWidth\":2,\"parentID\":1,\"port\":1,\"signalID\":229,\"signalName\":\"MATLAB Function1:1\"},\"type\":\"RecordBlkView.Signal\",\"uuid\":\"\"},{\"content\":{\"blockPath\":[],\"channel\":[229,1],\"dimensions\":[360,1],\"domain\":\"\",\"lineColor\":\"#b746ff\",\"lineWidth\":2,\"parentID\":1,\"port\":1,\"signalID\":230,\"signalName\":\"MATLAB Function1:1\"},\"type\":\"RecordBlkView.Signal\",\"uuid\":\"\"},{\"content\":{\"blockPath\":[],\"channel\":[230,1],\"dimensions\":[360,1],\"domain\":\"\",\"lineColor\":\"#64d413\",\"lineWidth\":2,\"parentID\":1,\"port\":1,\"signalID\":231,\"signalName\":\"MATLAB Function1:1\"},\"type\":\"RecordBlkView.Signal\",\"uuid\":\"\"},{\"content\":{\"blockPath\":[],\"channel\":[231,1],\"dimensions\":[360,1],\"domain\":\"\",\"lineColor\":\"#ff13a6\",\"lineWidth\":2,\"parentID\":1,\"port\":1,\"signalID\":232,\"signalName\":\"MATLAB Function1:1\"},\"type\":\"RecordBlkView.Signal\",\"uuid\":\"\"},{\"content\":{\"blockPath\":[],\"channel\":[232,1],\"dimensions\":[360,1],\"domain\":\"\",\"lineColor\":\"#fe330a\",\"lineWidth\":2,\"parentID\":1,\"port\":1,\"signalID\":233,\"signalName\":\"MATLAB Function1:1\"},\"type\":\"RecordBlkView.Signal\",\"uuid\":\"\"},{\"content\":{\"blockPath\":[],\"channel\":[233,1],\"dimensions\":[360,1],\"domain\":\"\",\"lineColor\":\"#22b573\",\"lineWidth\":2,\"parentID\":1,\"port\":1,\"signalID\":234,\"signalName\":\"MATLAB Function1:1\"},\"type\":\"RecordBlkView.Signal\",\"uuid\":\"\"},{\"content\":{\"blockPath\":[],\"channel\":[234,1],\"dimensions\":[360,1],\"domain\":\"\",\"lineColor\":\"#0072bd\",\"lineWidth\":2,\"parentID\":1,\"port\":1,\"signalID\":235,\"signalName\":\"MATLAB Function1:1\"},\"type\":\"RecordBlkView.Signal\",\"uuid\":\"\"},{\"content\":{\"blockPath\":[],\"channel\":[235,1],\"dimensions\":[360,1],\"domain\":\"\",\"lineColor\":\"#d95319\",\"lineWidth\":2,\"parentID\":1,\"port\":1,\"signalID\":236,\"signalName\":\"MATLAB Function1:1\"},\"type\":\"RecordBlkView.Signal\",\"uuid\":\"\"},{\"content\":{\"blockPath\":[],\"channel\":[236,1],\"dimensions\":[360,1],\"domain\":\"\",\"lineColor\":\"#edb120\",\"lineWidth\":2,\"parentID\":1,\"port\":1,\"signalID\":237,\"signalName\":\"MATLAB Function1:1\"},\"type\":\"RecordBlkView.Signal\",\"uuid\":\"\"},{\"content\":{\"blockPath\":[],\"channel\":[237,1],\"dimensions\":[360,1],\"domain\":\"\",\"lineColor\":\"#7e2f8e\",\"lineWidth\":2,\"parentID\":1,\"port\":1,\"signalID\":238,\"signalName\":\"MATLAB Function1:1\"},\"type\":\"RecordBlkView.Signal\",\"uuid\":\"\"},{\"content\":{\"blockPath\":[],\"channel\":[238,1],\"dimensions\":[360,1],\"domain\":\"\",\"lineColor\":\"#77ac30\",\"lineWidth\":2,\"parentID\":1,\"port\":1,\"signalID\":239,\"signalName\":\"MATLAB Function1:1\"},\"type\":\"RecordBlkView.Signal\",\"uuid\":\"\"},{\"content\":{\"blockPath\":[],\"channel\":[239,1],\"dimensions\":[360,1],\"domain\":\"\",\"lineColor\":\"#4dbeee\",\"lineWidth\":2,\"parentID\":1,\"port\":1,\"signalID\":240,\"signalName\":\"MATLAB Function1:1\"},\"type\":\"RecordBlkView.Signal\",\"uuid\":\"\"},{\"content\":{\"blockPath\":[],\"channel\":[240,1],\"dimensions\":[360,1],\"domain\":\"\",\"lineColor\":\"#a2142f\",\"lineWidth\":2,\"parentID\":1,\"port\":1,\"signalID\":241,\"signalName\":\"MATLAB Function1:1\"},\"type\":\"RecordBlkView.Signal\",\"uuid\":\"\"},{\"content\":{\"blockPath\":[],\"channel\":[241,1],\"dimensions\":[360,1],\"domain\":\"\",\"lineColor\":\"#139fff\",\"lineWidth\":2,\"parentID\":1,\"port\":1,\"signalID\":242,\"signalName\":\"MATLAB Function1:1\"},\"type\":\"RecordBlkView.Signal\",\"uuid\":\"\"},{\"content\":{\"blockPath\":[],\"channel\":[242,1],\"dimensions\":[360,1],\"domain\":\"\",\"lineColor\":\"#ff6929\",\"lineWidth\":2,\"parentID\":1,\"port\":1,\"signalID\":243,\"signalName\":\"MATLAB Function1:1\"},\"type\":\"RecordBlkView.Signal\",\"uuid\":\"\"},{\"content\":{\"blockPath\":[],\"channel\":[243,1],\"dimensions\":[360,1],\"domain\":\"\",\"lineColor\":\"#b746ff\",\"lineWidth\":2,\"parentID\":1,\"port\":1,\"signalID\":244,\"signalName\":\"MATLAB Function1:1\"},\"type\":\"RecordBlkView.Signal\",\"uuid\":\"\"},{\"content\":{\"blockPath\":[],\"channel\":[244,1],\"dimensions\":[360,1],\"domain\":\"\",\"lineColor\":\"#64d413\",\"lineWidth\":2,\"parentID\":1,\"port\":1,\"signalID\":245,\"signalName\":\"MATLAB Function1:1\"},\"type\":\"RecordBlkView.Signal\",\"uuid\":\"\"},{\"content\":{\"blockPath\":[],\"channel\":[245,1],\"dimensions\":[360,1],\"domain\":\"\",\"lineColor\":\"#ff13a6\",\"lineWidth\":2,\"parentID\":1,\"port\":1,\"signalID\":246,\"signalName\":\"MATLAB Function1:1\"},\"type\":\"RecordBlkView.Signal\",\"uuid\":\"\"},{\"content\":{\"blockPath\":[],\"channel\":[246,1],\"dimensions\":[360,1],\"domain\":\"\",\"lineColor\":\"#fe330a\",\"lineWidth\":2,\"parentID\":1,\"port\":1,\"signalID\":247,\"signalName\":\"MATLAB Function1:1\"},\"type\":\"RecordBlkView.Signal\",\"uuid\":\"\"},{\"content\":{\"blockPath\":[],\"channel\":[247,1],\"dimensions\":[360,1],\"domain\":\"\",\"lineColor\":\"#22b573\",\"lineWidth\":2,\"parentID\":1,\"port\":1,\"signalID\":248,\"signalName\":\"MATLAB Function1:1\"},\"type\":\"RecordBlkView.Signal\",\"uuid\":\"\"},{\"content\":{\"blockPath\":[],\"channel\":[248,1],\"dimensions\":[360,1],\"domain\":\"\",\"lineColor\":\"#0072bd\",\"lineWidth\":2,\"parentID\":1,\"port\":1,\"signalID\":249,\"signalName\":\"MATLAB Function1:1\"},\"type\":\"RecordBlkView.Signal\",\"uuid\":\"\"},{\"content\":{\"blockPath\":[],\"channel\":[249,1],\"dimensions\":[360,1],\"domain\":\"\",\"lineColor\":\"#d95319\",\"lineWidth\":2,\"parentID\":1,\"port\":1,\"signalID\":250,\"signalName\":\"MATLAB Function1:1\"},\"type\":\"RecordBlkView.Signal\",\"uuid\":\"\"},{\"content\":{\"blockPath\":[],\"channel\":[250,1],\"dimensions\":[360,1],\"domain\":\"\",\"lineColor\":\"#edb120\",\"lineWidth\":2,\"parentID\":1,\"port\":1,\"signalID\":251,\"signalName\":\"MATLAB Function1:1\"},\"type\":\"RecordBlkView.Signal\",\"uuid\":\"\"},{\"content\":{\"blockPath\":[],\"channel\":[251,1],\"dimensions\":[360,1],\"domain\":\"\",\"lineColor\":\"#7e2f8e\",\"lineWidth\":2,\"parentID\":1,\"port\":1,\"signalID\":252,\"signalName\":\"MATLAB Function1:1\"},\"type\":\"RecordBlkView.Signal\",\"uuid\":\"\"},{\"content\":{\"blockPath\":[],\"channel\":[252,1],\"dimensions\":[360,1],\"domain\":\"\",\"lineColor\":\"#77ac30\",\"lineWidth\":2,\"parentID\":1,\"port\":1,\"signalID\":253,\"signalName\":\"MATLAB Function1:1\"},\"type\":\"RecordBlkView.Signal\",\"uuid\":\"\"},{\"content\":{\"blockPath\":[],\"channel\":[253,1],\"dimensions\":[360,1],\"domain\":\"\",\"lineColor\":\"#4dbeee\",\"lineWidth\":2,\"parentID\":1,\"port\":1,\"signalID\":254,\"signalName\":\"MATLAB Function1:1\"},\"type\":\"RecordBlkView.Signal\",\"uuid\":\"\"},{\"content\":{\"blockPath\":[],\"channel\":[254,1],\"dimensions\":[360,1],\"domain\":\"\",\"lineColor\":\"#a2142f\",\"lineWidth\":2,\"parentID\":1,\"port\":1,\"signalID\":255,\"signalName\":\"MATLAB Function1:1\"},\"type\":\"RecordBlkView.Signal\",\"uuid\":\"\"},{\"content\":{\"blockPath\":[],\"channel\":[255,1],\"dimensions\":[360,1],\"domain\":\"\",\"lineColor\":\"#139fff\",\"lineWidth\":2,\"parentID\":1,\"port\":1,\"signalID\":256,\"signalName\":\"MATLAB Function1:1\"},\"type\":\"RecordBlkView.Signal\",\"uuid\":\"\"},{\"content\":{\"blockPath\":[],\"channel\":[256,1],\"dimensions\":[360,1],\"domain\":\"\",\"lineColor\":\"#ff6929\",\"lineWidth\":2,\"parentID\":1,\"port\":1,\"signalID\":257,\"signalName\":\"MATLAB Function1:1\"},\"type\":\"RecordBlkView.Signal\",\"uuid\":\"\"},{\"content\":{\"blockPath\":[],\"channel\":[257,1],\"dimensions\":[360,1],\"domain\":\"\",\"lineColor\":\"#b746ff\",\"lineWidth\":2,\"parentID\":1,\"port\":1,\"signalID\":258,\"signalName\":\"MATLAB Function1:1\"},\"type\":\"RecordBlkView.Signal\",\"uuid\":\"\"},{\"content\":{\"blockPath\":[],\"channel\":[258,1],\"dimensions\":[360,1],\"domain\":\"\",\"lineColor\":\"#64d413\",\"lineWidth\":2,\"parentID\":1,\"port\":1,\"signalID\":259,\"signalName\":\"MATLAB Function1:1\"},\"type\":\"RecordBlkView.Signal\",\"uuid\":\"\"},{\"content\":{\"blockPath\":[],\"channel\":[259,1],\"dimensions\":[360,1],\"domain\":\"\",\"lineColor\":\"#ff13a6\",\"lineWidth\":2,\"parentID\":1,\"port\":1,\"signalID\":260,\"signalName\":\"MATLAB Function1:1\"},\"type\":\"RecordBlkView.Signal\",\"uuid\":\"\"},{\"content\":{\"blockPath\":[],\"channel\":[260,1],\"dimensions\":[360,1],\"domain\":\"\",\"lineColor\":\"#fe330a\",\"lineWidth\":2,\"parentID\":1,\"port\":1,\"signalID\":261,\"signalName\":\"MATLAB Function1:1\"},\"type\":\"RecordBlkView.Signal\",\"uuid\":\"\"},{\"content\":{\"blockPath\":[],\"channel\":[261,1],\"dimensions\":[360,1],\"domain\":\"\",\"lineColor\":\"#22b573\",\"lineWidth\":2,\"parentID\":1,\"port\":1,\"signalID\":262,\"signalName\":\"MATLAB Function1:1\"},\"type\":\"RecordBlkView.Signal\",\"uuid\":\"\"},{\"content\":{\"blockPath\":[],\"channel\":[262,1],\"dimensions\":[360,1],\"domain\":\"\",\"lineColor\":\"#0072bd\",\"lineWidth\":2,\"parentID\":1,\"port\":1,\"signalID\":263,\"signalName\":\"MATLAB Function1:1\"},\"type\":\"RecordBlkView.Signal\",\"uuid\":\"\"},{\"content\":{\"blockPath\":[],\"channel\":[263,1],\"dimensions\":[360,1],\"domain\":\"\",\"lineColor\":\"#d95319\",\"lineWidth\":2,\"parentID\":1,\"port\":1,\"signalID\":264,\"signalName\":\"MATLAB Function1:1\"},\"type\":\"RecordBlkView.Signal\",\"uuid\":\"\"},{\"content\":{\"blockPath\":[],\"channel\":[264,1],\"dimensions\":[360,1],\"domain\":\"\",\"lineColor\":\"#edb120\",\"lineWidth\":2,\"parentID\":1,\"port\":1,\"signalID\":265,\"signalName\":\"MATLAB Function1:1\"},\"type\":\"RecordBlkView.Signal\",\"uuid\":\"\"},{\"content\":{\"blockPath\":[],\"channel\":[265,1],\"dimensions\":[360,1],\"domain\":\"\",\"lineColor\":\"#7e2f8e\",\"lineWidth\":2,\"parentID\":1,\"port\":1,\"signalID\":266,\"signalName\":\"MATLAB Function1:1\"},\"type\":\"RecordBlkView.Signal\",\"uuid\":\"\"},{\"content\":{\"blockPath\":[],\"channel\":[266,1],\"dimensions\":[360,1],\"domain\":\"\",\"lineColor\":\"#77ac30\",\"lineWidth\":2,\"parentID\":1,\"port\":1,\"signalID\":267,\"signalName\":\"MATLAB Function1:1\"},\"type\":\"RecordBlkView.Signal\",\"uuid\":\"\"},{\"content\":{\"blockPath\":[],\"channel\":[267,1],\"dimensions\":[360,1],\"domain\":\"\",\"lineColor\":\"#4dbeee\",\"lineWidth\":2,\"parentID\":1,\"port\":1,\"signalID\":268,\"signalName\":\"MATLAB Function1:1\"},\"type\":\"RecordBlkView.Signal\",\"uuid\":\"\"},{\"content\":{\"blockPath\":[],\"channel\":[268,1],\"dimensions\":[360,1],\"domain\":\"\",\"lineColor\":\"#a2142f\",\"lineWidth\":2,\"parentID\":1,\"port\":1,\"signalID\":269,\"signalName\":\"MATLAB Function1:1\"},\"type\":\"RecordBlkView.Signal\",\"uuid\":\"\"},{\"content\":{\"blockPath\":[],\"channel\":[269,1],\"dimensions\":[360,1],\"domain\":\"\",\"lineColor\":\"#139fff\",\"lineWidth\":2,\"parentID\":1,\"port\":1,\"signalID\":270,\"signalName\":\"MATLAB Function1:1\"},\"type\":\"RecordBlkView.Signal\",\"uuid\":\"\"},{\"content\":{\"blockPath\":[],\"channel\":[270,1],\"dimensions\":[360,1],\"domain\":\"\",\"lineColor\":\"#ff6929\",\"lineWidth\":2,\"parentID\":1,\"port\":1,\"signalID\":271,\"signalName\":\"MATLAB Function1:1\"},\"type\":\"RecordBlkView.Signal\",\"uuid\":\"\"},{\"content\":{\"blockPath\":[],\"channel\":[271,1],\"dimensions\":[360,1],\"domain\":\"\",\"lineColor\":\"#b746ff\",\"lineWidth\":2,\"parentID\":1,\"port\":1,\"signalID\":272,\"signalName\":\"MATLAB Function1:1\"},\"type\":\"RecordBlkView.Signal\",\"uuid\":\"\"},{\"content\":{\"blockPath\":[],\"channel\":[272,1],\"dimensions\":[360,1],\"domain\":\"\",\"lineColor\":\"#64d413\",\"lineWidth\":2,\"parentID\":1,\"port\":1,\"signalID\":273,\"signalName\":\"MATLAB Function1:1\"},\"type\":\"RecordBlkView.Signal\",\"uuid\":\"\"},{\"content\":{\"blockPath\":[],\"channel\":[273,1],\"dimensions\":[360,1],\"domain\":\"\",\"lineColor\":\"#ff13a6\",\"lineWidth\":2,\"parentID\":1,\"port\":1,\"signalID\":274,\"signalName\":\"MATLAB Function1:1\"},\"type\":\"RecordBlkView.Signal\",\"uuid\":\"\"},{\"content\":{\"blockPath\":[],\"channel\":[274,1],\"dimensions\":[360,1],\"domain\":\"\",\"lineColor\":\"#fe330a\",\"lineWidth\":2,\"parentID\":1,\"port\":1,\"signalID\":275,\"signalName\":\"MATLAB Function1:1\"},\"type\":\"RecordBlkView.Signal\",\"uuid\":\"\"},{\"content\":{\"blockPath\":[],\"channel\":[275,1],\"dimensions\":[360,1],\"domain\":\"\",\"lineColor\":\"#22b573\",\"lineWidth\":2,\"parentID\":1,\"port\":1,\"signalID\":276,\"signalName\":\"MATLAB Function1:1\"},\"type\":\"RecordBlkView.Signal\",\"uuid\":\"\"},{\"content\":{\"blockPath\":[],\"channel\":[276,1],\"dimensions\":[360,1],\"domain\":\"\",\"lineColor\":\"#0072bd\",\"lineWidth\":2,\"parentID\":1,\"port\":1,\"signalID\":277,\"signalName\":\"MATLAB Function1:1\"},\"type\":\"RecordBlkView.Signal\",\"uuid\":\"\"},{\"content\":{\"blockPath\":[],\"channel\":[277,1],\"dimensions\":[360,1],\"domain\":\"\",\"lineColor\":\"#d95319\",\"lineWidth\":2,\"parentID\":1,\"port\":1,\"signalID\":278,\"signalName\":\"MATLAB Function1:1\"},\"type\":\"RecordBlkView.Signal\",\"uuid\":\"\"},{\"content\":{\"blockPath\":[],\"channel\":[278,1],\"dimensions\":[360,1],\"domain\":\"\",\"lineColor\":\"#edb120\",\"lineWidth\":2,\"parentID\":1,\"port\":1,\"signalID\":279,\"signalName\":\"MATLAB Function1:1\"},\"type\":\"RecordBlkView.Signal\",\"uuid\":\"\"},{\"content\":{\"blockPath\":[],\"channel\":[279,1],\"dimensions\":[360,1],\"domain\":\"\",\"lineColor\":\"#7e2f8e\",\"lineWidth\":2,\"parentID\":1,\"port\":1,\"signalID\":280,\"signalName\":\"MATLAB Function1:1\"},\"type\":\"RecordBlkView.Signal\",\"uuid\":\"\"},{\"content\":{\"blockPath\":[],\"channel\":[280,1],\"dimensions\":[360,1],\"domain\":\"\",\"lineColor\":\"#77ac30\",\"lineWidth\":2,\"parentID\":1,\"port\":1,\"signalID\":281,\"signalName\":\"MATLAB Function1:1\"},\"type\":\"RecordBlkView.Signal\",\"uuid\":\"\"},{\"content\":{\"blockPath\":[],\"channel\":[281,1],\"dimensions\":[360,1],\"domain\":\"\",\"lineColor\":\"#4dbeee\",\"lineWidth\":2,\"parentID\":1,\"port\":1,\"signalID\":282,\"signalName\":\"MATLAB Function1:1\"},\"type\":\"RecordBlkView.Signal\",\"uuid\":\"\"},{\"content\":{\"blockPath\":[],\"channel\":[282,1],\"dimensions\":[360,1],\"domain\":\"\",\"lineColor\":\"#a2142f\",\"lineWidth\":2,\"parentID\":1,\"port\":1,\"signalID\":283,\"signalName\":\"MATLAB Function1:1\"},\"type\":\"RecordBlkView.Signal\",\"uuid\":\"\"},{\"content\":{\"blockPath\":[],\"channel\":[283,1],\"dimensions\":[360,1],\"domain\":\"\",\"lineColor\":\"#139fff\",\"lineWidth\":2,\"parentID\":1,\"port\":1,\"signalID\":284,\"signalName\":\"MATLAB Function1:1\"},\"type\":\"RecordBlkView.Signal\",\"uuid\":\"\"},{\"content\":{\"blockPath\":[],\"channel\":[284,1],\"dimensions\":[360,1],\"domain\":\"\",\"lineColor\":\"#ff6929\",\"lineWidth\":2,\"parentID\":1,\"port\":1,\"signalID\":285,\"signalName\":\"MATLAB Function1:1\"},\"type\":\"RecordBlkView.Signal\",\"uuid\":\"\"},{\"content\":{\"blockPath\":[],\"channel\":[285,1],\"dimensions\":[360,1],\"domain\":\"\",\"lineColor\":\"#b746ff\",\"lineWidth\":2,\"parentID\":1,\"port\":1,\"signalID\":286,\"signalName\":\"MATLAB Function1:1\"},\"type\":\"RecordBlkView.Signal\",\"uuid\":\"\"},{\"content\":{\"blockPath\":[],\"channel\":[286,1],\"dimensions\":[360,1],\"domain\":\"\",\"lineColor\":\"#64d413\",\"lineWidth\":2,\"parentID\":1,\"port\":1,\"signalID\":287,\"signalName\":\"MATLAB Function1:1\"},\"type\":\"RecordBlkView.Signal\",\"uuid\":\"\"},{\"content\":{\"blockPath\":[],\"channel\":[287,1],\"dimensions\":[360,1],\"domain\":\"\",\"lineColor\":\"#ff13a6\",\"lineWidth\":2,\"parentID\":1,\"port\":1,\"signalID\":288,\"signalName\":\"MATLAB Function1:1\"},\"type\":\"RecordBlkView.Signal\",\"uuid\":\"\"},{\"content\":{\"blockPath\":[],\"channel\":[288,1],\"dimensions\":[360,1],\"domain\":\"\",\"lineColor\":\"#fe330a\",\"lineWidth\":2,\"parentID\":1,\"port\":1,\"signalID\":289,\"signalName\":\"MATLAB Function1:1\"},\"type\":\"RecordBlkView.Signal\",\"uuid\":\"\"},{\"content\":{\"blockPath\":[],\"channel\":[289,1],\"dimensions\":[360,1],\"domain\":\"\",\"lineColor\":\"#22b573\",\"lineWidth\":2,\"parentID\":1,\"port\":1,\"signalID\":290,\"signalName\":\"MATLAB Function1:1\"},\"type\":\"RecordBlkView.Signal\",\"uuid\":\"\"},{\"content\":{\"blockPath\":[],\"channel\":[290,1],\"dimensions\":[360,1],\"domain\":\"\",\"lineColor\":\"#0072bd\",\"lineWidth\":2,\"parentID\":1,\"port\":1,\"signalID\":291,\"signalName\":\"MATLAB Function1:1\"},\"type\":\"RecordBlkView.Signal\",\"uuid\":\"\"},{\"content\":{\"blockPath\":[],\"channel\":[291,1],\"dimensions\":[360,1],\"domain\":\"\",\"lineColor\":\"#d95319\",\"lineWidth\":2,\"parentID\":1,\"port\":1,\"signalID\":292,\"signalName\":\"MATLAB Function1:1\"},\"type\":\"RecordBlkView.Signal\",\"uuid\":\"\"},{\"content\":{\"blockPath\":[],\"channel\":[292,1],\"dimensions\":[360,1],\"domain\":\"\",\"lineColor\":\"#edb120\",\"lineWidth\":2,\"parentID\":1,\"port\":1,\"signalID\":293,\"signalName\":\"MATLAB Function1:1\"},\"type\":\"RecordBlkView.Signal\",\"uuid\":\"\"},{\"content\":{\"blockPath\":[],\"channel\":[293,1],\"dimensions\":[360,1],\"domain\":\"\",\"lineColor\":\"#7e2f8e\",\"lineWidth\":2,\"parentID\":1,\"port\":1,\"signalID\":294,\"signalName\":\"MATLAB Function1:1\"},\"type\":\"RecordBlkView.Signal\",\"uuid\":\"\"},{\"content\":{\"blockPath\":[],\"channel\":[294,1],\"dimensions\":[360,1],\"domain\":\"\",\"lineColor\":\"#77ac30\",\"lineWidth\":2,\"parentID\":1,\"port\":1,\"signalID\":295,\"signalName\":\"MATLAB Function1:1\"},\"type\":\"RecordBlkView.Signal\",\"uuid\":\"\"},{\"content\":{\"blockPath\":[],\"channel\":[295,1],\"dimensions\":[360,1],\"domain\":\"\",\"lineColor\":\"#4dbeee\",\"lineWidth\":2,\"parentID\":1,\"port\":1,\"signalID\":296,\"signalName\":\"MATLAB Function1:1\"},\"type\":\"RecordBlkView.Signal\",\"uuid\":\"\"},{\"content\":{\"blockPath\":[],\"channel\":[296,1],\"dimensions\":[360,1],\"domain\":\"\",\"lineColor\":\"#a2142f\",\"lineWidth\":2,\"parentID\":1,\"port\":1,\"signalID\":297,\"signalName\":\"MATLAB Function1:1\"},\"type\":\"RecordBlkView.Signal\",\"uuid\":\"\"},{\"content\":{\"blockPath\":[],\"channel\":[297,1],\"dimensions\":[360,1],\"domain\":\"\",\"lineColor\":\"#139fff\",\"lineWidth\":2,\"parentID\":1,\"port\":1,\"signalID\":298,\"signalName\":\"MATLAB Function1:1\"},\"type\":\"RecordBlkView.Signal\",\"uuid\":\"\"},{\"content\":{\"blockPath\":[],\"channel\":[298,1],\"dimensions\":[360,1],\"domain\":\"\",\"lineColor\":\"#ff6929\",\"lineWidth\":2,\"parentID\":1,\"port\":1,\"signalID\":299,\"signalName\":\"MATLAB Function1:1\"},\"type\":\"RecordBlkView.Signal\",\"uuid\":\"\"},{\"content\":{\"blockPath\":[],\"channel\":[299,1],\"dimensions\":[360,1],\"domain\":\"\",\"lineColor\":\"#b746ff\",\"lineWidth\":2,\"parentID\":1,\"port\":1,\"signalID\":300,\"signalName\":\"MATLAB Function1:1\"},\"type\":\"RecordBlkView.Signal\",\"uuid\":\"\"},{\"content\":{\"blockPath\":[],\"channel\":[300,1],\"dimensions\":[360,1],\"domain\":\"\",\"lineColor\":\"#64d413\",\"lineWidth\":2,\"parentID\":1,\"port\":1,\"signalID\":301,\"signalName\":\"MATLAB Function1:1\"},\"type\":\"RecordBlkView.Signal\",\"uuid\":\"\"},{\"content\":{\"blockPath\":[],\"channel\":[301,1],\"dimensions\":[360,1],\"domain\":\"\",\"lineColor\":\"#ff13a6\",\"lineWidth\":2,\"parentID\":1,\"port\":1,\"signalID\":302,\"signalName\":\"MATLAB Function1:1\"},\"type\":\"RecordBlkView.Signal\",\"uuid\":\"\"},{\"content\":{\"blockPath\":[],\"channel\":[302,1],\"dimensions\":[360,1],\"domain\":\"\",\"lineColor\":\"#fe330a\",\"lineWidth\":2,\"parentID\":1,\"port\":1,\"signalID\":303,\"signalName\":\"MATLAB Function1:1\"},\"type\":\"RecordBlkView.Signal\",\"uuid\":\"\"},{\"content\":{\"blockPath\":[],\"channel\":[303,1],\"dimensions\":[360,1],\"domain\":\"\",\"lineColor\":\"#22b573\",\"lineWidth\":2,\"parentID\":1,\"port\":1,\"signalID\":304,\"signalName\":\"MATLAB Function1:1\"},\"type\":\"RecordBlkView.Signal\",\"uuid\":\"\"},{\"content\":{\"blockPath\":[],\"channel\":[304,1],\"dimensions\":[360,1],\"domain\":\"\",\"lineColor\":\"#0072bd\",\"lineWidth\":2,\"parentID\":1,\"port\":1,\"signalID\":305,\"signalName\":\"MATLAB Function1:1\"},\"type\":\"RecordBlkView.Signal\",\"uuid\":\"\"},{\"content\":{\"blockPath\":[],\"channel\":[305,1],\"dimensions\":[360,1],\"domain\":\"\",\"lineColor\":\"#d95319\",\"lineWidth\":2,\"parentID\":1,\"port\":1,\"signalID\":306,\"signalName\":\"MATLAB Function1:1\"},\"type\":\"RecordBlkView.Signal\",\"uuid\":\"\"},{\"content\":{\"blockPath\":[],\"channel\":[306,1],\"dimensions\":[360,1],\"domain\":\"\",\"lineColor\":\"#edb120\",\"lineWidth\":2,\"parentID\":1,\"port\":1,\"signalID\":307,\"signalName\":\"MATLAB Function1:1\"},\"type\":\"RecordBlkView.Signal\",\"uuid\":\"\"},{\"content\":{\"blockPath\":[],\"channel\":[307,1],\"dimensions\":[360,1],\"domain\":\"\",\"lineColor\":\"#7e2f8e\",\"lineWidth\":2,\"parentID\":1,\"port\":1,\"signalID\":308,\"signalName\":\"MATLAB Function1:1\"},\"type\":\"RecordBlkView.Signal\",\"uuid\":\"\"},{\"content\":{\"blockPath\":[],\"channel\":[308,1],\"dimensions\":[360,1],\"domain\":\"\",\"lineColor\":\"#77ac30\",\"lineWidth\":2,\"parentID\":1,\"port\":1,\"signalID\":309,\"signalName\":\"MATLAB Function1:1\"},\"type\":\"RecordBlkView.Signal\",\"uuid\":\"\"},{\"content\":{\"blockPath\":[],\"channel\":[309,1],\"dimensions\":[360,1],\"domain\":\"\",\"lineColor\":\"#4dbeee\",\"lineWidth\":2,\"parentID\":1,\"port\":1,\"signalID\":310,\"signalName\":\"MATLAB Function1:1\"},\"type\":\"RecordBlkView.Signal\",\"uuid\":\"\"},{\"content\":{\"blockPath\":[],\"channel\":[310,1],\"dimensions\":[360,1],\"domain\":\"\",\"lineColor\":\"#a2142f\",\"lineWidth\":2,\"parentID\":1,\"port\":1,\"signalID\":311,\"signalName\":\"MATLAB Function1:1\"},\"type\":\"RecordBlkView.Signal\",\"uuid\":\"\"},{\"content\":{\"blockPath\":[],\"channel\":[311,1],\"dimensions\":[360,1],\"domain\":\"\",\"lineColor\":\"#139fff\",\"lineWidth\":2,\"parentID\":1,\"port\":1,\"signalID\":312,\"signalName\":\"MATLAB Function1:1\"},\"type\":\"RecordBlkView.Signal\",\"uuid\":\"\"},{\"content\":{\"blockPath\":[],\"channel\":[312,1],\"dimensions\":[360,1],\"domain\":\"\",\"lineColor\":\"#ff6929\",\"lineWidth\":2,\"parentID\":1,\"port\":1,\"signalID\":313,\"signalName\":\"MATLAB Function1:1\"},\"type\":\"RecordBlkView.Signal\",\"uuid\":\"\"},{\"content\":{\"blockPath\":[],\"channel\":[313,1],\"dimensions\":[360,1],\"domain\":\"\",\"lineColor\":\"#b746ff\",\"lineWidth\":2,\"parentID\":1,\"port\":1,\"signalID\":314,\"signalName\":\"MATLAB Function1:1\"},\"type\":\"RecordBlkView.Signal\",\"uuid\":\"\"},{\"content\":{\"blockPath\":[],\"channel\":[314,1],\"dimensions\":[360,1],\"domain\":\"\",\"lineColor\":\"#64d413\",\"lineWidth\":2,\"parentID\":1,\"port\":1,\"signalID\":315,\"signalName\":\"MATLAB Function1:1\"},\"type\":\"RecordBlkView.Signal\",\"uuid\":\"\"},{\"content\":{\"blockPath\":[],\"channel\":[315,1],\"dimensions\":[360,1],\"domain\":\"\",\"lineColor\":\"#ff13a6\",\"lineWidth\":2,\"parentID\":1,\"port\":1,\"signalID\":316,\"signalName\":\"MATLAB Function1:1\"},\"type\":\"RecordBlkView.Signal\",\"uuid\":\"\"},{\"content\":{\"blockPath\":[],\"channel\":[316,1],\"dimensions\":[360,1],\"domain\":\"\",\"lineColor\":\"#fe330a\",\"lineWidth\":2,\"parentID\":1,\"port\":1,\"signalID\":317,\"signalName\":\"MATLAB Function1:1\"},\"type\":\"RecordBlkView.Signal\",\"uuid\":\"\"},{\"content\":{\"blockPath\":[],\"channel\":[317,1],\"dimensions\":[360,1],\"domain\":\"\",\"lineColor\":\"#22b573\",\"lineWidth\":2,\"parentID\":1,\"port\":1,\"signalID\":318,\"signalName\":\"MATLAB Function1:1\"},\"type\":\"RecordBlkView.Signal\",\"uuid\":\"\"},{\"content\":{\"blockPath\":[],\"channel\":[318,1],\"dimensions\":[360,1],\"domain\":\"\",\"lineColor\":\"#0072bd\",\"lineWidth\":2,\"parentID\":1,\"port\":1,\"signalID\":319,\"signalName\":\"MATLAB Function1:1\"},\"type\":\"RecordBlkView.Signal\",\"uuid\":\"\"},{\"content\":{\"blockPath\":[],\"channel\":[319,1],\"dimensions\":[360,1],\"domain\":\"\",\"lineColor\":\"#d95319\",\"lineWidth\":2,\"parentID\":1,\"port\":1,\"signalID\":320,\"signalName\":\"MATLAB Function1:1\"},\"type\":\"RecordBlkView.Signal\",\"uuid\":\"\"},{\"content\":{\"blockPath\":[],\"channel\":[320,1],\"dimensions\":[360,1],\"domain\":\"\",\"lineColor\":\"#edb120\",\"lineWidth\":2,\"parentID\":1,\"port\":1,\"signalID\":321,\"signalName\":\"MATLAB Function1:1\"},\"type\":\"RecordBlkView.Signal\",\"uuid\":\"\"},{\"content\":{\"blockPath\":[],\"channel\":[321,1],\"dimensions\":[360,1],\"domain\":\"\",\"lineColor\":\"#7e2f8e\",\"lineWidth\":2,\"parentID\":1,\"port\":1,\"signalID\":322,\"signalName\":\"MATLAB Function1:1\"},\"type\":\"RecordBlkView.Signal\",\"uuid\":\"\"},{\"content\":{\"blockPath\":[],\"channel\":[322,1],\"dimensions\":[360,1],\"domain\":\"\",\"lineColor\":\"#77ac30\",\"lineWidth\":2,\"parentID\":1,\"port\":1,\"signalID\":323,\"signalName\":\"MATLAB Function1:1\"},\"type\":\"RecordBlkView.Signal\",\"uuid\":\"\"},{\"content\":{\"blockPath\":[],\"channel\":[323,1],\"dimensions\":[360,1],\"domain\":\"\",\"lineColor\":\"#4dbeee\",\"lineWidth\":2,\"parentID\":1,\"port\":1,\"signalID\":324,\"signalName\":\"MATLAB Function1:1\"},\"type\":\"RecordBlkView.Signal\",\"uuid\":\"\"},{\"content\":{\"blockPath\":[],\"channel\":[324,1],\"dimensions\":[360,1],\"domain\":\"\",\"lineColor\":\"#a2142f\",\"lineWidth\":2,\"parentID\":1,\"port\":1,\"signalID\":325,\"signalName\":\"MATLAB Function1:1\"},\"type\":\"RecordBlkView.Signal\",\"uuid\":\"\"},{\"content\":{\"blockPath\":[],\"channel\":[325,1],\"dimensions\":[360,1],\"domain\":\"\",\"lineColor\":\"#139fff\",\"lineWidth\":2,\"parentID\":1,\"port\":1,\"signalID\":326,\"signalName\":\"MATLAB Function1:1\"},\"type\":\"RecordBlkView.Signal\",\"uuid\":\"\"},{\"content\":{\"blockPath\":[],\"channel\":[326,1],\"dimensions\":[360,1],\"domain\":\"\",\"lineColor\":\"#ff6929\",\"lineWidth\":2,\"parentID\":1,\"port\":1,\"signalID\":327,\"signalName\":\"MATLAB Function1:1\"},\"type\":\"RecordBlkView.Signal\",\"uuid\":\"\"},{\"content\":{\"blockPath\":[],\"channel\":[327,1],\"dimensions\":[360,1],\"domain\":\"\",\"lineColor\":\"#b746ff\",\"lineWidth\":2,\"parentID\":1,\"port\":1,\"signalID\":328,\"signalName\":\"MATLAB Function1:1\"},\"type\":\"RecordBlkView.Signal\",\"uuid\":\"\"},{\"content\":{\"blockPath\":[],\"channel\":[328,1],\"dimensions\":[360,1],\"domain\":\"\",\"lineColor\":\"#64d413\",\"lineWidth\":2,\"parentID\":1,\"port\":1,\"signalID\":329,\"signalName\":\"MATLAB Function1:1\"},\"type\":\"RecordBlkView.Signal\",\"uuid\":\"\"},{\"content\":{\"blockPath\":[],\"channel\":[329,1],\"dimensions\":[360,1],\"domain\":\"\",\"lineColor\":\"#ff13a6\",\"lineWidth\":2,\"parentID\":1,\"port\":1,\"signalID\":330,\"signalName\":\"MATLAB Function1:1\"},\"type\":\"RecordBlkView.Signal\",\"uuid\":\"\"},{\"content\":{\"blockPath\":[],\"channel\":[330,1],\"dimensions\":[360,1],\"domain\":\"\",\"lineColor\":\"#fe330a\",\"lineWidth\":2,\"parentID\":1,\"port\":1,\"signalID\":331,\"signalName\":\"MATLAB Function1:1\"},\"type\":\"RecordBlkView.Signal\",\"uuid\":\"\"},{\"content\":{\"blockPath\":[],\"channel\":[331,1],\"dimensions\":[360,1],\"domain\":\"\",\"lineColor\":\"#22b573\",\"lineWidth\":2,\"parentID\":1,\"port\":1,\"signalID\":332,\"signalName\":\"MATLAB Function1:1\"},\"type\":\"RecordBlkView.Signal\",\"uuid\":\"\"},{\"content\":{\"blockPath\":[],\"channel\":[332,1],\"dimensions\":[360,1],\"domain\":\"\",\"lineColor\":\"#0072bd\",\"lineWidth\":2,\"parentID\":1,\"port\":1,\"signalID\":333,\"signalName\":\"MATLAB Function1:1\"},\"type\":\"RecordBlkView.Signal\",\"uuid\":\"\"},{\"content\":{\"blockPath\":[],\"channel\":[333,1],\"dimensions\":[360,1],\"domain\":\"\",\"lineColor\":\"#d95319\",\"lineWidth\":2,\"parentID\":1,\"port\":1,\"signalID\":334,\"signalName\":\"MATLAB Function1:1\"},\"type\":\"RecordBlkView.Signal\",\"uuid\":\"\"},{\"content\":{\"blockPath\":[],\"channel\":[334,1],\"dimensions\":[360,1],\"domain\":\"\",\"lineColor\":\"#edb120\",\"lineWidth\":2,\"parentID\":1,\"port\":1,\"signalID\":335,\"signalName\":\"MATLAB Function1:1\"},\"type\":\"RecordBlkView.Signal\",\"uuid\":\"\"},{\"content\":{\"blockPath\":[],\"channel\":[335,1],\"dimensions\":[360,1],\"domain\":\"\",\"lineColor\":\"#7e2f8e\",\"lineWidth\":2,\"parentID\":1,\"port\":1,\"signalID\":336,\"signalName\":\"MATLAB Function1:1\"},\"type\":\"RecordBlkView.Signal\",\"uuid\":\"\"},{\"content\":{\"blockPath\":[],\"channel\":[336,1],\"dimensions\":[360,1],\"domain\":\"\",\"lineColor\":\"#77ac30\",\"lineWidth\":2,\"parentID\":1,\"port\":1,\"signalID\":337,\"signalName\":\"MATLAB Function1:1\"},\"type\":\"RecordBlkView.Signal\",\"uuid\":\"\"},{\"content\":{\"blockPath\":[],\"channel\":[337,1],\"dimensions\":[360,1],\"domain\":\"\",\"lineColor\":\"#4dbeee\",\"lineWidth\":2,\"parentID\":1,\"port\":1,\"signalID\":338,\"signalName\":\"MATLAB Function1:1\"},\"type\":\"RecordBlkView.Signal\",\"uuid\":\"\"},{\"content\":{\"blockPath\":[],\"channel\":[338,1],\"dimensions\":[360,1],\"domain\":\"\",\"lineColor\":\"#a2142f\",\"lineWidth\":2,\"parentID\":1,\"port\":1,\"signalID\":339,\"signalName\":\"MATLAB Function1:1\"},\"type\":\"RecordBlkView.Signal\",\"uuid\":\"\"},{\"content\":{\"blockPath\":[],\"channel\":[339,1],\"dimensions\":[360,1],\"domain\":\"\",\"lineColor\":\"#139fff\",\"lineWidth\":2,\"parentID\":1,\"port\":1,\"signalID\":340,\"signalName\":\"MATLAB Function1:1\"},\"type\":\"RecordBlkView.Signal\",\"uuid\":\"\"},{\"content\":{\"blockPath\":[],\"channel\":[340,1],\"dimensions\":[360,1],\"domain\":\"\",\"lineColor\":\"#ff6929\",\"lineWidth\":2,\"parentID\":1,\"port\":1,\"signalID\":341,\"signalName\":\"MATLAB Function1:1\"},\"type\":\"RecordBlkView.Signal\",\"uuid\":\"\"},{\"content\":{\"blockPath\":[],\"channel\":[341,1],\"dimensions\":[360,1],\"domain\":\"\",\"lineColor\":\"#b746ff\",\"lineWidth\":2,\"parentID\":1,\"port\":1,\"signalID\":342,\"signalName\":\"MATLAB Function1:1\"},\"type\":\"RecordBlkView.Signal\",\"uuid\":\"\"},{\"content\":{\"blockPath\":[],\"channel\":[342,1],\"dimensions\":[360,1],\"domain\":\"\",\"lineColor\":\"#64d413\",\"lineWidth\":2,\"parentID\":1,\"port\":1,\"signalID\":343,\"signalName\":\"MATLAB Function1:1\"},\"type\":\"RecordBlkView.Signal\",\"uuid\":\"\"},{\"content\":{\"blockPath\":[],\"channel\":[343,1],\"dimensions\":[360,1],\"domain\":\"\",\"lineColor\":\"#ff13a6\",\"lineWidth\":2,\"parentID\":1,\"port\":1,\"signalID\":344,\"signalName\":\"MATLAB Function1:1\"},\"type\":\"RecordBlkView.Signal\",\"uuid\":\"\"},{\"content\":{\"blockPath\":[],\"channel\":[344,1],\"dimensions\":[360,1],\"domain\":\"\",\"lineColor\":\"#fe330a\",\"lineWidth\":2,\"parentID\":1,\"port\":1,\"signalID\":345,\"signalName\":\"MATLAB Function1:1\"},\"type\":\"RecordBlkView.Signal\",\"uuid\":\"\"},{\"content\":{\"blockPath\":[],\"channel\":[345,1],\"dimensions\":[360,1],\"domain\":\"\",\"lineColor\":\"#22b573\",\"lineWidth\":2,\"parentID\":1,\"port\":1,\"signalID\":346,\"signalName\":\"MATLAB Function1:1\"},\"type\":\"RecordBlkView.Signal\",\"uuid\":\"\"},{\"content\":{\"blockPath\":[],\"channel\":[346,1],\"dimensions\":[360,1],\"domain\":\"\",\"lineColor\":\"#0072bd\",\"lineWidth\":2,\"parentID\":1,\"port\":1,\"signalID\":347,\"signalName\":\"MATLAB Function1:1\"},\"type\":\"RecordBlkView.Signal\",\"uuid\":\"\"},{\"content\":{\"blockPath\":[],\"channel\":[347,1],\"dimensions\":[360,1],\"domain\":\"\",\"lineColor\":\"#d95319\",\"lineWidth\":2,\"parentID\":1,\"port\":1,\"signalID\":348,\"signalName\":\"MATLAB Function1:1\"},\"type\":\"RecordBlkView.Signal\",\"uuid\":\"\"},{\"content\":{\"blockPath\":[],\"channel\":[348,1],\"dimensions\":[360,1],\"domain\":\"\",\"lineColor\":\"#edb120\",\"lineWidth\":2,\"parentID\":1,\"port\":1,\"signalID\":349,\"signalName\":\"MATLAB Function1:1\"},\"type\":\"RecordBlkView.Signal\",\"uuid\":\"\"},{\"content\":{\"blockPath\":[],\"channel\":[349,1],\"dimensions\":[360,1],\"domain\":\"\",\"lineColor\":\"#7e2f8e\",\"lineWidth\":2,\"parentID\":1,\"port\":1,\"signalID\":350,\"signalName\":\"MATLAB Function1:1\"},\"type\":\"RecordBlkView.Signal\",\"uuid\":\"\"},{\"content\":{\"blockPath\":[],\"channel\":[350,1],\"dimensions\":[360,1],\"domain\":\"\",\"lineColor\":\"#77ac30\",\"lineWidth\":2,\"parentID\":1,\"port\":1,\"signalID\":351,\"signalName\":\"MATLAB Function1:1\"},\"type\":\"RecordBlkView.Signal\",\"uuid\":\"\"},{\"content\":{\"blockPath\":[],\"channel\":[351,1],\"dimensions\":[360,1],\"domain\":\"\",\"lineColor\":\"#4dbeee\",\"lineWidth\":2,\"parentID\":1,\"port\":1,\"signalID\":352,\"signalName\":\"MATLAB Function1:1\"},\"type\":\"RecordBlkView.Signal\",\"uuid\":\"\"},{\"content\":{\"blockPath\":[],\"channel\":[352,1],\"dimensions\":[360,1],\"domain\":\"\",\"lineColor\":\"#a2142f\",\"lineWidth\":2,\"parentID\":1,\"port\":1,\"signalID\":353,\"signalName\":\"MATLAB Function1:1\"},\"type\":\"RecordBlkView.Signal\",\"uuid\":\"\"},{\"content\":{\"blockPath\":[],\"channel\":[353,1],\"dimensions\":[360,1],\"domain\":\"\",\"lineColor\":\"#139fff\",\"lineWidth\":2,\"parentID\":1,\"port\":1,\"signalID\":354,\"signalName\":\"MATLAB Function1:1\"},\"type\":\"RecordBlkView.Signal\",\"uuid\":\"\"},{\"content\":{\"blockPath\":[],\"channel\":[354,1],\"dimensions\":[360,1],\"domain\":\"\",\"lineColor\":\"#ff6929\",\"lineWidth\":2,\"parentID\":1,\"port\":1,\"signalID\":355,\"signalName\":\"MATLAB Function1:1\"},\"type\":\"RecordBlkView.Signal\",\"uuid\":\"\"},{\"content\":{\"blockPath\":[],\"channel\":[355,1],\"dimensions\":[360,1],\"domain\":\"\",\"lineColor\":\"#b746ff\",\"lineWidth\":2,\"parentID\":1,\"port\":1,\"signalID\":356,\"signalName\":\"MATLAB Function1:1\"},\"type\":\"RecordBlkView.Signal\",\"uuid\":\"\"},{\"content\":{\"blockPath\":[],\"channel\":[356,1],\"dimensions\":[360,1],\"domain\":\"\",\"lineColor\":\"#64d413\",\"lineWidth\":2,\"parentID\":1,\"port\":1,\"signalID\":357,\"signalName\":\"MATLAB Function1:1\"},\"type\":\"RecordBlkView.Signal\",\"uuid\":\"\"},{\"content\":{\"blockPath\":[],\"channel\":[357,1],\"dimensions\":[360,1],\"domain\":\"\",\"lineColor\":\"#ff13a6\",\"lineWidth\":2,\"parentID\":1,\"port\":1,\"signalID\":358,\"signalName\":\"MATLAB Function1:1\"},\"type\":\"RecordBlkView.Signal\",\"uuid\":\"\"},{\"content\":{\"blockPath\":[],\"channel\":[358,1],\"dimensions\":[360,1],\"domain\":\"\",\"lineColor\":\"#fe330a\",\"lineWidth\":2,\"parentID\":1,\"port\":1,\"signalID\":359,\"signalName\":\"MATLAB Function1:1\"},\"type\":\"RecordBlkView.Signal\",\"uuid\":\"\"},{\"content\":{\"blockPath\":[],\"channel\":[359,1],\"dimensions\":[360,1],\"domain\":\"\",\"lineColor\":\"#22b573\",\"lineWidth\":2,\"parentID\":1,\"port\":1,\"signalID\":360,\"signalName\":\"MATLAB Function1:1\"},\"type\":\"RecordBlkView.Signal\",\"uuid\":\"\"},{\"content\":{\"blockPath\":[],\"channel\":[360,1],\"dimensions\":[360,1],\"domain\":\"\",\"lineColor\":\"#0072bd\",\"lineWidth\":2,\"parentID\":1,\"port\":1,\"signalID\":361,\"signalName\":\"MATLAB Function1:1\"},\"type\":\"RecordBlkView.Signal\",\"uuid\":\"\"},{\"content\":{\"blockPath\":[],\"dimensions\":[360,1],\"domain\":\"\",\"hasChildren\":true,\"lineColor\":\"#7e2f8e\",\"lineWidth\":2,\"port\":2,\"signalID\":362,\"signalName\":\"MATLAB Function1:2\"},\"type\":\"RecordBlkView.Signal\",\"uuid\":\"\"},{\"content\":{\"blockPath\":[],\"channel\":[1,1],\"dimensions\":[360,1],\"domain\":\"\",\"lineColor\":\"#77ac30\",\"lineWidth\":2,\"parentID\":362,\"port\":2,\"signalID\":363,\"signalName\":\"MATLAB Function1:2\"},\"type\":\"RecordBlkView.Signal\",\"uuid\":\"\"}]},\"type\":\"RecordBlkView.InputSignals\",\"uuid\":\"\"}],\"packageUris\":[\"http:\\/\\/schema.mathworks.com\\/mf0\\/streamout_blocks\\/R2020a\"],\"version\":\"1.0\"}"  VisualizationBindings="{\"xyplotplugin\":{\"info\":[{\"series\":[{\"bindingParametersList\":[{\"parameter\":\"X-Axis\",\"signalID\":363,\"signalName\":\"MATLAB Function1:2\"},{\"parameter\":\"Y-Axis\",\"signalID\":363,\"signalName\":\"MATLAB Function1:2\"}],\"seriesID\":0},{\"bindingParametersList\":[{\"parameter\":\"X-Axis\",\"signalID\":363,\"signalName\":\"MATLAB Function1:2\"},{\"parameter\":\"Y-Axis\",\"signalID\":363,\"signalName\":\"MATLAB Function1:2\"}],\"seriesID\":1},{\"bindingParametersList\":[{\"parameter\":\"X-Axis\",\"signalID\":2,\"signalName\":\"MATLAB Function1:1(1,1)\"},{\"parameter\":\"Y-Axis\",\"signalID\":2,\"signalName\":\"MATLAB Function1:1(1,1)\"}],\"seriesID\":2}],\"subplotID\":1}]}}"  CompatibilityTag=XY
  carrot_method : MATLAB Function  TreatAsAtomicUnit=on
  wires:
  Subscribe1/2 -> Bus Selector3/1
  Subscribe1/1 -> Proportional Controller1/Enable, Command Velocity Publisher/Enable  "IsNew"
  Bus Selector3/1 -> Command Velocity Publisher/1(header)  "<header>"
  Bus Selector3/4 -> MATLAB Function/1(qx)  "<x>"
  Bus Selector3/5 -> MATLAB Function/2(qy)  "<y>"
  Bus Selector3/6 -> MATLAB Function/3(qz)  "<z>"
  Bus Selector3/7 -> MATLAB Function/4(qw)  "<w>"
  Subscribe2/2 -> Bus Selector/1
  Bus Selector/1 -> MATLAB Function1/1(ranges), carrot_method/4(ranges)  "<ranges>"
  Bus Selector3/2 -> MATLAB Function1/4(pose_x), Proportional Controller1/2(Position X), carrot_method/1(pose_x), XY Graph/1  "<x>"
  Bus Selector3/3 -> MATLAB Function1/5(pose_y), carrot_method/2(pose_y), Proportional Controller1/3(Position Y), XY Graph/2  "<y>"
  Bus Selector/2 -> MATLAB Function1/2(angle_min), carrot_method/5(angle_min)  "<angle_min>"
  Bus Selector/4 -> MATLAB Function1/3(angle_inc), carrot_method/6(angle_inc)  "<angle_increment>"
  MATLAB Function/1(theta) -> carrot_method/3(pose_theta), MATLAB Function1/6(pose_theta), Proportional Controller1/4(Orientation (theta))
  Proportional Controller1/2(Angular Velocity (w)) -> MATLAB Function1/7(angular_vel), Command Velocity Publisher/3(w)
  Proportional Controller1/1(Linear Velocity (v)) -> Command Velocity Publisher/2(v)
  carrot_method/1(target_x) -> Mux/1
  carrot_method/2(target_y) -> Mux/2
  Mux/1 -> Proportional Controller1/1(Desired position)
  Bus Selector/3 -> ?  "<angle_max>"
